simulink model "ASM_Traffic_A11"  (R2026a)
settings: Solver=ode1  StartTime=SIM.tstart.v  StopTime=SIM.tend.v  FixedStep=SIM.StepSize.v
PostLoadFcn:
  | if any(exist('dsrtsu_mdlpostloadfcn', 'file') ~= 0), dsrtsu_mdlpostloadfcn('Execute', bdroot); end
  | try, asm_mdl_postloadfcn(bdroot, 'UpdateModel', 3600); catch, disp(lasterr); end,
InitFcn:
  | , if any(exist('rtifpga_mdlclblib', 'file') ~= 0), rtifpga_mdlclblib('Init', bdroot); end,
  | , if any(exist('dsmpb_private', 'file') ~= 0), dsmpb_private('dsmpb_mdlclblib', 'Init', bdroot); end,
undefined symbols (not defined in the file): _to_, a0b2, ASM_BrakeHydraulics_DemoSystems, ASM_VehicleDynamics_DemoSystems, b98103fe8ad365046cd0, BrakeCircuit, controllerConfig, CPT, Crankshaft, DiscIntNeverNeededParam, dsmsi, FinalDriveAssembly, instance, MDL, ModeSignals, mu, Pos_BrakePedal_Maneuver, rad, RefSignals, s_to_rpm, SIM, SoftECU, Suspension, Tire, Transmission
libraries: ASM_Traffic_lib x135, simulink x98, ASM_Utils_lib x77, ASM_VehicleDynamics_lib x70, ASM_Environment_lib x22, dsmpblib x20, dsmsilib x15, MDLD_Utils_lib x10, ASM_BrakeHydraulics_lib x3, sl_discontinuities x2
(part 1 of 63)
PreSaveFcn:
  | , if any(exist('dsmpb_private', 'file') ~= 0), dsmpb_private('dsmpb_mdlclblib', 'PreSave', bdroot); end,
CloseFcn:
  | , if any(exist('dsmpb_private', 'file') ~= 0), dsmpb_private('dsmpb_mdlclblib', 'Close', bdroot); end,
settings Model: DataDictionary=vehicle_control.sldd  RTICANMMDATA=struct('GeneralSetupData',struct('modelroot','C:\_GIT\ASM\Demo\Traffic\Sources\Simulation\Models','generalsettings',struct('filesettings',struct('destfolder',struct('Name','RTICANMM_FILES','Check',1),'buildfolder',struct('Name','.','Check',1),'AbsDestfolder',struct('Name','C:\_GIT\ASM\Demo\Traffic\Sources\Simulation\Models\RTICANMM_FILES'),'AbsBuildfolder',struct('Name','C:\_GIT\ASM\Demo\Traffic\Sources\Simulation\Models'))),'options',struct('addpaths',1,'rmpaths',1,'addtrcexclusion',true,'cannavigator',struct('checkmonitoring',0),'show_usrtrc',0,'use_usrtrc',0),'advanced',struct('options',ones(1,100)),'MPSetup',{{}},'RTI',struct('Type','DSRT','Ver','4.5','Date','02-May-2021'),'modelname','ASM_Traffic','block','ASM_Traffic'))  RTILINMMDATA=struct('GeneralSetupData',[])  DSRTSU_INTERNAL_MDBS_VER=10  DSRTSU_INTERNAL_FLEXRAYCONFIG=1  DSRTSU_INTERNAL_RTIFPGA=231  DSPACE_VER=struct('Name',{['Aerospace Blockset'],['Aerospace Toolbox'],['Communications System Toolbox'],['Control System Toolbox'],['DSP System Toolbox'],['Fixed-Point Designer'],['Fuzzy Logic Toolbox'],'MATLAB',['MATLAB Coder'],['MATLAB Report Generator'],['Neural Network Toolbox'],['Optimization Toolbox'],['Robust Control Toolbox'],['Signal Processing Toolbox'],'SimMechanics','SimPowerSystems','Simscape','Simulink',['Simulink Coder'],['Simulink Control Design'],['Simulink Report Generator'],['Spreadsheet Link EX'],'Stateflow',['System Identification Toolbox'],['dSPACE APU_Table_Modification_Library'],['dSPACE AnalogSingleChannelLibrary'],['dSPACE Automotive Simulation Models'],['dSPACE BCE-HILBlockset'],['dSPACE BitLibrary'],['dSPACE BuildHelperLibrary'],['dSPACE BusLoadMeasurementBlockset'],['dSPACE ByteStreamLibrary'],['dSPACE CANObserver'],['dSPACE CANUtilLibrary'],['dSPACE DS5337RSimBlockset'],['dSPACE DS5381InterfaceBlockset'],['dSPACE DSMSU'],['dSPACE DiagnosticTester'],['dSPACE DynamicTrc'],['dSPACE ENGLibrary'],['dSPACE ESPLibrary'],['dSPACE FIUDS291ControlBlockset'],['dSPACE FlexRay Configuration Blockset'],['dSPACE FlexRayModelBuilder'],['dSPACE IOBlocksLibrary'],['dSPACE InfoBlock'],['dSPACE LabelInterface'],['dSPACE LibsDependencyHelper'],['dSPACE MATLAB Connection'],['dSPACE MATLAB Integration Main'],['dSPACE MatlabApplToolsSingleSetupBaseScripts'],['dSPACE Model Port Block Library'],['dSPACE Model Separation Block Library'],['dSPACE MotionDesk Blockset'],['dSPACE MultiSignalTa'],['dSPACE PWMLibrary'],['dSPACE RTCANModules'],['dSPACE RTI Bypass Blockset'],['dSPACE RTI CAN Blockset'],['dSPACE RTI CAN MultiMessage Blockset'],['dSPACE RTI EMC Blockset'],['dSPACE RTI ETHERNET Blockset'],['dSPACE RTI ETHERNETUDP Blockset'],['dSPACE RTI FPGA Programming Blockset'],['dSPACE RTI FlexRay Configuration Blockset'],['dSPACE RTI Gigalink Blockset'],['dSPACE RTI LIN MultiMessage Blockset'],['dSPACE RTI MultiMessage Shared Utilities'],['dSPACE RTI RPCU Blockset'],['dSPACE RTI USBFLIGHTREC Blockset'],['dSPACE RTI WATCHDOG Blockset'],['dSPACE RTI XCP on Ethernet Blockset'],['dSPACE RTI for Multiprocessor Systems RTI-MP'],['dSPACE Real-Time Interface (RTI1006)'],['dSPACE Real-Time Interface Shared Utilities'],['dSPACE Run-Time Target'],['dSPACE Run-Time Target Shared Utilities'],['dSPACE SCLibrary'],['dSPACE SENTLibrary'],['dSPACE ScalingLibrary'],['dSPACE SignalLibrary'],['dSPACE SpeedSensorLibrary'],['dSPACE StructureBrowser'],['dSPACE TALib'],['dSPACE UtilitiesGUI'],['dSPACE VariationHandling'],['dSPACE XILMapper']},'Version',{'3.16','2.16','6.1','9.10','9.1','5.1','2.2.22','8.6','3.0','4.2','8.4','7.3','6.0','7.1','4.7','6.4','3.14','8.6','8.9','4.2.1','4.2','3.2.4','8.6','9.3','1.5','1.29','8.4','15.1.0.5','2.7.6','1.3.10','1.12','1.7.1','1.5.7','2.7.4','1.4.7.1','3.7.2','2.13','1.16','5.1.7','2.8.9','2.7.4','2.6.20','2.9','1.78','2.6.6','1.1.8','8.2.0.10','1.0','2.4','2.2','1.5','3.4','3.4','2.5.1','2.3.1','2.6.6','4.3.33','3.8','3.4.4','4.5','1.4','1.2.2','1.4.2','3.3','3.9','2.3.2','2.8','1.9.4','2.2.2','1.2.1','2.1','1.2.9','7.8','7.8','7.8','3.4','3.3','2.25','1.83','2.0','2.8.6','2.9.10','3.1','2.64','2.44','8.3.5','1.4'},'Release',{'(R2015b)','(R2015b)','(R2015b)','(R2015b)','(R2015b)','(R2015b)','(R2015b)','(R2015b)','(R2015b)','(R2015b)','(R2015b)','(R2015b)','(R2015b)','(R2015b)','(R2015b)','(R2015b)','(R2015b)','(R2015b)','(R2015b)','(R2015b)','(R2015b)','(R2015b)','(R2015b)','(R2015b)','','','','','','','','','','','','','','','','','','','','','','','','','','','','','','','','','','','','','','','','','','','','','','','','','','','','','','','','','','','','','','',''},'Date',{'13-Aug-2015','13-Aug-2015','13-Aug-2015','13-Aug-2015','13-Aug-2015','13-Aug-2015','13-Aug-2015','13-Aug-2015','13-Aug-2015','13-Aug-2015','13-Aug-2015','13-Aug-2015','13-Aug-2015','13-Aug-2015','13-Aug-2015','13-Aug-2015','13-Aug-2015','13-Aug-2015','13-Aug-2015','13-Aug-2015','13-Aug-2015','13-Aug-2015','13-Aug-2015','13-Aug-2015','14-Jul-2017','14-Jul-2017','02-May-2017','26-Jul-2017','26-Jul-2017','14-Jul-2017','14-Jul-2017','26-Jul-2017','14-Jul-2017','14-Jul-2017','26-Jul-2017','21-Jul-2017','14-Jul-2017','14-Jul-2017','14-Jul-2017','14-Jul-2017','14-Jul-2017','14-Jul-2017','02-May-2017','14-Jul-2017','14-Jul-2017','14-Jul-2017','14-Jul-2017','14-Jul-2017','01-Jun-2012','02-Nov-2017','11-Sep-2017','02-May-2017','02-May-2017','02-May-2017','26-Jul-2017','26-Jul-2017','21-Aug-2017','02-May-2017','02-May-2017','02-May-2017','02-May-2017','02-May-2017','02-May-2017','02-May-2017','02-May-2016','02-May-2017','02-May-2017','02-May-2017','02-May-2017','02-May-2017','02-May-2017','02-May-2017','02-May-2017','02-May-2017','02-May-2017','02-May-2017','02-May-2016','14-Jul-2017','14-Jul-2017','23-Aug-2017','14-Jul-2017','14-Jul-2017','14-Jul-2017','24-Jul-2017','14-Jul-2017','30-Aug-2017','14-Jul-2017'})  DSMPB_DATASERVER_ModelPortLibVersion1=8  DSMPB_DATASERVER_DataServerVersion1=6  DSMPB_DATASERVER_DataServerStreamVersion1=3  DSRTSU_INTERNAL_RTISTBM_VER=26.1  DSMPB_ID_DATA={'800713',struct('BlockId','12fb6bc3-5111-44d0-a4e3-361b98a9a776','SignalIds',{{'026ddceb-0771-416e-9843-dcd8d1431538','61e2bdca-47a9-456d-99cd-a85121b8e8fe','d0b83999-293c-421a-8719-21ab1d67d0de','ee79a2a1-d570-4cea-bcdb-c9b139602f90','57ea1fa1-ca61-4546-b593-c63adff471df','4745b4fa-0f34-4fbf-be5c-f27e4134315a','de5a6e89-ccb7-4a59-b515-490b9b995fd4','ad253b40-3f00-490f-9ecf-d815cc0cc36e','cc49b837-b150-45e5-8f90-c3d0e2d27081','b15d69de-ed07-4862-a514-9609c89542f8','13fce408-6e36-44ee-bb67-08a7b0eb2fa4','0f4551f6-6300-456d-9d9a-57c69ec52a7f','d36d9585-c1d8-4a20-931e-65168d3abe38','f057ce8d-e313-4b61-85c9-b9b6cfbd35a4','6c11160e-2f21-4e5c-9a52-ebbb9f762535','e6450135-026d-470e-aadb-d378b73b5a20','d236869c-3852-4609-804f-fcde24edb3a3','dc22ee5e-8ec6-4b0e-aea7-12268f14ea36','758aa22a-c1dd-488c-99a3-602f258deef7','bc79a9cd-46f9-40fa-919c-8e2738391b36','ebfaacba-c463-48d7-b1a3-39c653a8c3db','464c7844-6639-4bb4-8711-079b53f28673','4c39bdf6-9afd-4077-adbf-78dbe8d90694','d3194eeb-2c4d-4fae-92b4-da69ec7b3ff0','1db3a7e8-3ac4-49c7-9bab-9691ec783862','90ff480f-e2cd-45c5-a9e2-c8c85a7416d4','f175cdee-a16d-4d06-b6b9-468792d9fc63','5037e91f-c007-4d18-9ed3-e85dcdcb817d','365a1b2d-a520-4285-8b7d-0710eb545db2','ad84fb44-ff2d-41bf-b3fb-6e536509c574','949ac335-20f1-4cbb-bd1f-899e13a3e7a3','821ab1d9-2030-4fa0-bc2e-dfd2cf9be3b6','b9c006ab-bd85-4d65-a229-7e38f2547f6c','555683a2-7050-45d2-912c-54f0995d7ba8','92371cf3-d090-4109-a430-860de30ac424','353c2b7d-88ed-484a-861a-3a12ddecabcf','5b259f8e-4f91-45a6-a068-ded45fefdcc6','01be563f-388e-4058-a34f-f6cfb35f92e8','924754af-4079-4771-ade8-70a8e93fbf63','6cf2dfc4-e3af-4f2a-86ef-faba7990cd7d','6c53c97e-f8d9-411f-9845-8d7d23140d3b'}}),'800714',struct('BlockId','c8c3f793-af41-48c0-af0b-d118a4506f01','SignalIds',{{'9a85b6de-5177-4fe9-a45c-5ce81acce6a0','07d402bb-9325-4ff2-835b-9988c7203a47','e23e99f8-e557-4f94-a0a8-73349e51b7d3','1e2029dd-c64a-4f77-920a-b53592f4df24','79f5377a-112c-44fb-95ad-b93421afa7d0','fab0e021-301d-4150-96e9-7c18ce36f7d6'}}),'800715',struct('BlockId','64fe778b-45c6-4580-ad77-0b0bfacf3090','SignalIds',{{'c4b7fff6-f5fb-46b8-aa58-6d02b0742f95','1b507cb2-f8a9-4150-a5ca-84f7e7defee9','0800db64-ae10-48a7-b8a4-d98403852f64','7b5be15e-1bb0-4f29-a798-1f0dfb3c643b','55455eeb-e67c-459e-83e8-a412efa38a5a'}}),'800716',struct('BlockId','110f2d64-38d9-4620-a52f-7bcb09150783','SignalIds',{{'378c6c24-c180-4551-b7dd-c3d67f95d979','8fbebc1f-626e-4f60-8692-ff751c91aa77','6c7a7005-bb3b-414b-8b4c-d96ebde91b51','fd069fef-3f82-419a-9093-61a227734c9d','43ee6e1a-a539-4eeb-8eea-2974459fcd70','b309ea5b-cecf-423c-8781-a1d200972b1c','ae18cdd8-d414-48f9-9705-1c32113b2bf5','a47b08e9-bc20-43f2-89f9-f6ef5b9b9052','d52309de-83ba-4b81-be00-3c772a7db2e7'}}),'800717',struct('BlockId','2899132d-e1ca-416b-8f40-193c3fe897ac','SignalIds',{{'0be58094-6177-48f8-a93d-65142150c1e5','0ecd58d0-6214-4a37-a63e-4304fffa59de','4e270858-0fe5-4a89-ae3c-f92717842777','7564fa9e-cfd4-4df7-85ff-40634c98855f','f1470ea9-9cad-48c1-ae87-969ea9d571ca','5b5bebc5-776f-4a59-bf41-42658f78f728','a2387763-f235-471c-8654-38e764b051d8','461d803a-6400-4d45-8627-c36525a15027','2aea000e-ed67-4eb5-bd93-f8c260051b4c','cbf9e4cd-e9c3-4c64-ae9b-53aeb7b537f4','2b8362d7-cb62-4e81-889e-7432047b1611','d9a94446-b01b-42e7-9a12-b8e6590ad696','8d0f7580-69d3-4b5c-9a99-fd9213d24abb','8100021c-0ed4-4fa9-8bda-2d5f13b5b25c','739ab445-ce00-41fa-b359-832193f86cf1','d8540c08-79a2-4101-8769-084a7d989adb','0456d1da-e15d-4f84-b42f-5f0d6692b1d6','05a518bf-3959-41e8-bc6c-520d23ad1964','a3f23e7d-f547-4381-9f96-2cf61720eb8e','b0dffef0-6031-4ae9-aedd-823f4c618df3','ad3989a0-e252-44d2-9a0c-04f71baba5bc','ceeb7a50-52ea-4ea4-9007-a364fa77e3c6','c1f783be-9b03-4e5f-bdd5-bb8170b1d4e8','c1ec2c99-3048-450a-b67a-74422a158205','92235c85-c9cc-4b2e-9e84-fcab8cbdacf5','65d7570b-7e96-4496-a46b-2ced650781d8','6a8ce03d-0951-45fc-b3eb-05c2cd91d985','a6c24270-e0ee-4c37-a87c-804f6f78e6a6','dcbe338a-832a-4956-b7eb-6f217ad8bffd','f3d6ffb2-cf2a-4737-8562-4466766efd81','e3fc5c7f-9c10-4ed4-b3a5-3afb283b4064','6d1ed271-15a9-4450-a3ba-f7bb57f64ead','a8ba92dc-13bf-4092-8674-9e191bb7156d','c7354c00-bb0a-4e0e-9409-06a293ddd3c8','0eb2deca-de7b-4d2b-aef4-e4c396decc62','1a679372-da5c-4f17-b380-c6a2bf11d2c1','9ab79166-e826-4110-a0c4-535e2d710ca8','390f325e-bb6c-4962-9120-8a4300e0738e','be43b800-7928-44f2-a4c0-456242549674','94810d38-2474-4cca-8aed-c3c732d73dfb','a3c555d4-b57b-442c-bc5f-42b549e0ebdd','fa686c6f-57fa-4a19-8654-6bb0d89b9d8b','317fafc6-aa92-42fc-af4b-7e632b8dd6cb','42f758a5-2c9e-4e81-9e7f-7d05391bf3b4','95628c4c-8a2d-45d6-9031-c67e967b97bd','053040ee-7507-481d-9488-55c16059fd65','321ce886-d869-4a8c-ad53-a1182d7ebf7f','2f696ce9-8e82-4494-85b6-6edf41a524ba','96c19483-5db4-47db-b22f-cb8f6c71aaa7','4ab31462-1fe1-425e-9686-6c57800097be','abf784ea-ad12-4b9b-bc2e-530352b16490','38c309fa-99f7-46f8-8d6e-2b0e652896be','e8acec3c-5d72-4d22-a694-701a6e4415b0','1ff94e3c-5fa0-4134-8bb8-33777bace64e','9fc01bdf-7a2b-401a-9f97-847a1bae8365','382a0f0c-2480-4a75-9d5e-ae6ebdcc659a','4eb20648-628b-4e6f-ac33-2eeb9d126ccb'}}),'800718',struct('BlockId','c7b5bfe3-a6be-46ec-a50d-4aab3ffc24a9','SignalIds',{{'deb772d2-6c98-466a-af94-833c1e8c6a36','cec82f56-8cc7-4b94-b67a-0596894dbebe','6382e864-8515-4680-a048-db954d71ab26','91e981ed-2272-4996-ad40-8a28f4d6dd53','9d667ac4-4e72-44d2-8b3f-72ed78a704bd','b18fe58e-af28-4bce-959c-12f7f85ad0f3','3aa2c131-9c84-410c-98de-2fe01e4a908b','35507932-4bd5-48e2-9485-b375285d832d','cd5b9c3e-56c1-4d2b-9a1f-945395cc32d3','24eebe62-153d-4bce-a518-49c16cde84f5','4305de8d-f825-44f6-9ca5-0c7611fd522b','17e29716-ca54-48d0-bc62-5fe9f3434ca1','cd3b7b0f-c36d-4cbb-9379-f81b2c6784f8','58d80150-ba28-4376-9565-4f54e4772edb','c576d0a5-0790-4567-987c-cbe91a75f0ba','50664475-5b64-4e66-9f4b-73bc2fea1a6e','aac5ca77-fdc8-4e25-87c7-90ed104b35ab'}}),'800719',struct('BlockId','fd333250-5108-4bdd-b217-05742883b635','SignalIds',{{'fd6e4402-dbaf-4d1c-bd82-13425e573e08','80cd8a48-d5fe-43c4-94e8-1cb6116a8ed7','c93f02f4-8690-4b3f-aacf-dccb2e469f89','97a0d73a-2704-491b-baea-065e5044d9d2','84a2e8dc-aed6-489a-94c8-65c6b07fd9b8','dfadd777-133c-42ac-820c-b33d6acf198f','c486474c-f3c8-4087-9f03-9d730f82c385','beba5407-f372-4db7-a348-241e24965918','ad25fe6a-7c71-482a-8ce4-10e2b2982753','277316e0-b6ae-46e2-b77d-e820d153e69e','1f1ccb49-e040-4775-b555-ae961c45c1ad','f1e14c28-6f99-46e6-b62b-c3d342fb5443','91bc19e6-da3c-4265-aeed-a1989e826b66','47a757e7-3497-432a-a330-11ddc874cd64','8d6042c8-cd6d-42f3-b882-ae0739e92277','4cce8199-ae31-46ba-accf-bf53829b41f1','5635eaf9-a30a-4fc4-ae77-4cb5eca17a9d','ee61cb28-d577-487b-8d44-ca6116171fcf','e7ac0723-c0ce-428c-8c8c-067eeb8da74c','d1b53615-1e53-4ce2-b64f-38a5f7733f09','cdbdca06-6486-42aa-b430-cb4a52eea665','850a5dee-225f-478a-9581-615a2f48f7ad','854c96a0-0707-4b6b-b6f8-0a183b00e44e','b51f722a-63c8-4799-80f6-5869d1768c86','afacac09-78ed-4c28-afc3-caf5182c97e4','3838c120-da0f-43e6-8c82-f4acfe70f498','0ec37172-fd37-40de-a1a5-d592bab9638c','f6432d1b-9c84-4f2d-9c11-26b8895372d0','88cd5d72-dcf7-4fa2-aa1c-4defdddab07e','9e3d05f8-118b-44d4-bf73-9541a35eccb6','47c50691-23f2-4614-8d16-3486ef70962b','df1199db-e244-4ea3-ba3a-6d95e1d3ab35','d0e15ae8-1f1b-4aca-b5c1-25fd3bc4d7b1','943c66f4-642f-4813-83a4-aeced7a93800','a414337f-60a5-451c-85a6-1cf67a2bdc2a','47656cf3-7131-4a8b-8897-3d4f5ee504dc','19df50e1-62cc-41c2-a1ae-8a30072c1769','6313e6c4-800c-4bc6-b483-562a296c6696','253d101f-cf3f-48bb-8256-ca9e2c176994','842ccb91-7488-4424-a1bd-ee0dc5452e02','edfb4f2c-8887-4268-896b-d3d4cf08511f','be61a72f-860b-41f0-ae5f-29ebc26172cf','be000a67-2b4e-4015-b53e-1fbbf3a008ff','462755d8-e6d8-4a64-9626-426b47122f26','82c58b5b-69d7-4d8e-b402-7f1b4c1a700a','1e6d3f4b-3b03-470e-923b-22159f6cada5','5f049c30-bd46-49c7-ac48-7e1f6fefb530','a0e0b802-6f7f-49b7-a429-c48ca4d4139e','1281ac42-8e28-42c0-a936-4005a211601b','9beb0e9a-27d3-476a-9d13-99abe4cea843','f53d3867-dbef-4261-b1c3-2b4dee163be1','ee2aa355-4a17-444b-902a-772860eaddf1','32460b21-dccc-4b01-877e-a94aaf934646','863063ab-8cc2-4a40-b442-f9966cff8d6e','83f86310-1a7f-49e6-afc4-440052af8f12','47d5607d-3f4f-46ab-85b1-751519f5b805','08ed226f-598d-4aac-861b-044b7f32584c','4bd63bc5-4130-469e-8f22-d01f9f4fce98','ed130744-95a8-4396-98fd-6fdf7b74c868','d25515f7-636d-412b-a108-6469ece34014','e0a9f995-7fa2-47f3-a847-f9f484ba4f2c','b862dec0-72c0-4713-a690-404fc8b02f29','c3bb2c82-685d-49ae-b6af-b90687468879','afbaa59e-7f77-4310-971c-bae7947abc48','90602b8e-bb8c-4b0d-9b2b-c62ce4fdf7e7','1c856c8b-b541-4516-b46b-1f3d62cbbfe1','7cc261c0-4f47-4e61-8dd4-d78e25dbdecf','c7bc511e-0b65-4e98-9c9a-920064cb6b63','bfd1d56d-f13f-4e5e-823f-952e754dbd0c','82de7653-b024-4c13-8012-f38d758e9954','2b4044e1-44f2-4903-950b-be8ac8baacaf','0dd165a1-5364-4028-bd1a-b406b00946c2','2f264a39-d831-47f4-96bb-f9fe5ff30a53','9df5b4b7-db8f-4bdd-b4d5-9d6a9a0ffdb2','1a66a4ee-350e-4c2c-bf40-f022062406c2','77a18b2e-c672-4761-91dd-6eafa4e19102','12d51f03-4dbd-4ec6-83b2-f715a521a52a','7bf7b22e-517c-4b95-b2bf-97bfc99264dd','add68492-0910-453d-ab19-c30bda99b2c6','cbd58389-3dea-48d1-b9e1-406211fb2dab','e50a4cd7-600e-4355-bb15-3c094bcc5ac1','3a0447da-a263-4f93-93eb-0e9b9100edb0','912e2f1f-6f47-44d8-adcb-1b8177648d58','e486dd64-d6e8-437c-a6a0-b199f2efdb0e','d2ee6f75-3cb1-4eef-983b-ed71a6d1bb38','c1952aa1-b2a5-48c0-a2d0-942ec9e7f2f4','49bde967-5132-4542-89bd-c4654eefdd77','3be74dcc-f43c-45cf-b54a-b5c65f19a43b','818406ab-e94a-445d-b1b5-ba61124e00c4','8f71f621-8c70-4d64-a2c2-b488647126d4','4da05b13-dc65-4e7c-b1b9-878991124cbd','6e83efe6-c8f9-4231-92d4-b4d7f0668546','69993996-e1d1-496c-aca1-69ffe8fae1a5','84fc7653-5de2-48aa-8e1a-968f1166a742','258a0b8e-5f88-4752-9ab5-3c0b8ebda0b5','441ae18f-f8be-4dcd-b94f-7ba9930a13ac','21dfff82-3c2b-4ea9-91c7-dcce8ece5997','346f0f1d-f939-4453-a2d2-0dcb996e0a1e','a36adb97-89fe-4899-a265-6520c71b3ff5','813f486c-74f5-4eca-967f-6c42063ea4dd','c4d42689-f4f0-4b6f-a38e-f84d5d9356d5','b6f52c18-269e-4fbf-8d79-b3a8502dcf1d','be3be440-49a6-4e5e-a8ea-e101f1f97e46','1443e3c7-0b66-4559-9d5c-022bd6fb1413','3619d79d-62a1-40ad-8798-8aef318fc3c0','ccd1bc00-75bd-4940-86fd-cde09b68246b','4897e56f-50bc-4408-afa8-8836e69b4214','2a747099-ef0f-49a8-a673-c9e2bf0431a8','2a05c281-76dd-4b18-bdcc-8b0b1623de33','8e8b9e3d-9da6-4c91-ad97-da351e7c5ce4','3aa74a25-b846-475e-b85d-2bda7118e9fb','36e5d7cf-1e55-485d-9ea5-607404581b83','6e9c588c-5111-456f-8df5-7d28f79b85fd','11f87df0-b446-4532-a0da-a61e3f519a1b','eeb7ca53-14f3-48d3-8cbd-30d53393f24d','15cb62d6-efef-442c-9095-4a4daf8331f2','571764dd-0a10-437d-a524-f0b9ab7344e5','8b504bc9-b5c9-4e82-b1fa-78aea347ec15','998dad1e-5600-4381-ab22-e7f3f524ae7a','662aecf5-3045-45ca-b11e-e7d87e8d0b8a','b10085a7-b175-4d8c-b90f-2bc7d40414d6','f4edeeab-2a70-406a-b919-7fdbdd2abf9d','37caa2d2-32f1-4563-85cc-686b833a5474','f4833482-eca0-4dbe-8fa7-2a1e94c23c99','e51f2174-4775-4a15-a086-b4a7f7e75b6b','8d7a3b7c-fd97-47f2-8c27-22f6e203736d','e5956908-2186-4f10-ae9a-fd057fe70ff8','721d1792-f1e9-42b0-a3a2-0e3fa8e0e821','d2a202d4-6127-4e89-935c-9d92cdd87736','386fdbd0-531c-494b-8426-924329178d82','efe7a87d-9b97-4251-a568-6f0ca7f4e92c','1f7fa3b9-bbd9-405e-b404-8a9e18586bee','432e3bed-77cf-45a5-85cc-11e334fd07f8','86045c54-912a-407b-b67e-f78922ce536e','457cdd77-786f-48ea-b3b2-c3e03235aa0a','633e14cc-c11e-4ac1-a483-775611aea1c1','a258e7ad-81ee-4dea-b8be-6e7ac4e44621','4ef6a072-1e8b-47a5-b341-a5dcbcd8cb90','33a3ceb0-8ab8-44a3-a3d2-f71013987fea','c36f3052-c68e-4376-b40d-ddf2055ae487','75d2ad53-8848-47bc-b5d6-a7e0017612c5','bd5d9453-6739-4499-981d-84dd39093b80','969f387d-3fc8-407c-a5e5-028362e5a95b','f11fe3f3-e9fc-42ac-844b-205184b71153','499e8514-fefe-4d7a-b40c-ef24d59ba918','a8201869-cac4-4380-a59b-e6c9f75760dd','98eed4a8-86bc-4747-917b-86404f1357ed','e289c530-b7de-4f7a-959d-0126ecacaf5b','5e5aadde-87cb-43d4-9746-29a9e6093a01','eb12c2ea-8f65-44ff-b461-5fd33f643dd4','bb210c61-1ec1-4936-995b-6bbfc57ddf98','e18cb670-c569-458d-978c-40f8ce8be5d4','4fbc0806-ca61-49f6-aace-fe0dcaff62a6','e7b2d3a3-c8df-462f-baaa-a2d16ec68154','f460289b-3dc1-424c-921b-29a4e305af97','f7d7a98e-f960-4832-bed6-be5d87bc3939','ada121aa-b9e0-4352-af98-831065332c99','384a259e-8ab7-4f48-bcc5-2d9370d1f415','41a3b8e0-6640-407d-bac0-c67ec7bacf7f','76e3ba12-398d-4d52-8e72-77b36df0b8f9','cbf1e48a-45ea-4ed2-aac2-f30a6de77e52','5b48e4e9-cb2b-4d01-ad8c-9e091345c2c7','8f53c525-7b72-43d2-9700-c7f983d8bedf','1cc60d1e-b8ae-4cf8-8851-0c49bafae1ef','be881860-d9f9-47b3-9d26-2e8339e236fb','2f5214f4-3645-4631-9005-571891b6352d','2acd13c6-dc04-46ae-bbb2-6839e982ab9b','9c40bc30-58b7-4191-8583-d0a20298e448','673b273c-3b84-4498-8285-a0a40c19a0f4','f19513a3-3d55-4382-a04a-5103d5267d86','5b5d4cf0-5436-41ce-8909-db5899b0366b','34adf297-cc5d-493b-9e6a-f695daa8b49c','3ed04828-0fc0-4e22-bef2-0a837b1a85e6','10cc9fe1-d523-4eeb-b681-c0c9e714530f','651a801c-6def-4724-9352-2a0d2f461e9e','0df446cd-9d88-4826-bffc-e9c9dacefbfd','529d7a46-f3fe-4bbd-ba1f-0fa165edf0f1','839c4579-a867-4396-b3ce-b6ac5267bb63','4a4e2f74-833f-4f7f-a54b-0a013ee938dc','85878658-3eb9-44a1-ad3d-539db9b60dfd','b3bab6cb-b43a-4861-9cb4-d8e7e4b2477a','9e08f04f-1cd4-4178-acdf-28e3ba30a904','e170d6ef-c360-41ca-b395-23487890b9ba','26eff205-14b9-4985-b337-2ee8592d01ee','c5bd0156-31e4-4237-bae7-be3fbabb6203','19a317f3-6d6d-4b8d-be7d-2f7dd3f41750','124aebf3-3ce1-4170-a17f-7ca68554ecab','260553de-b45c-4d7a-9ccc-678cba5c894d','c193bf19-d2e3-496a-b007-3e21fac56152','cbc4fb28-7ad3-42de-b3ee-6295ec2f5ed3','28f39ef9-8949-4eb7-a170-43df15bf335d','61054bc3-cff2-4e79-bfde-bac599f810fa','e865ec6c-644e-4526-b712-0e2c4af0429c','32d97da3-463a-4a75-9f72-02b74bdc2bdc','88c36d39-a5f0-4d09-9904-1c7d2863a1e5','b034d8fc-249f-4dc5-92b7-0e3f3fdddb16','55809439-d5b0-440e-adf4-415722c7ff7d','ec6ba6c6-5833-4612-995a-d48b47c2f1f1','b6a9966d-13f7-4837-aa64-8ac9eb77e9fe','1d664ff5-9564-42f5-86ce-0d8c55423f0f','9f619f56-85ed-44e0-be73-a9b7045679b2','68285cc2-83af-4a99-aa80-754e09911ae7','11d1c7e3-e8cc-45ef-98ac-71242c47fd69','e3c649b7-6571-49f0-b0fb-7ed4a441295f','11e241bf-760a-480a-b056-0d8ea1b83eb2','5438b643-3610-43a0-b3da-962e8ccc3a6c','70645b38-5664-4bc9-820c-6fb34a07cf55','bf395dbf-7dc4-4a31-bab6-f5f2d09649ef','9b6ebebd-ce58-4762-809d-f61da916c82c','8e5c654b-aa01-460e-ab69-b31230631c49','5b25f867-2790-40d7-833f-efd4b524b300','d29247f7-3ac8-4f63-91df-421bb2412626','ea999d2b-b741-4245-97be-0568eb343541','ae6ce583-3c9d-424b-bd65-be44f01e3fe2','dfd20957-1c86-415b-98fc-03254081b7f9','d5258cd8-92b4-4d96-b282-a49a7bb033a4','91e5d8c9-c3be-40af-82a3-39f6fee7fd72','ade0190c-86e5-48c4-8cbc-94be3d179650','926c42aa-9323-4532-98b6-cbace0f916cd','815ed81a-3c7d-4cd2-8ddb-729019ad6a5d','96882bdd-5ef0-46ff-9e86-5f86cd211018','1b29f201-1d91-4a69-a201-e625071d402a','132ec7eb-3cb2-4b84-8dc9-c1b60432f37f','fefbfcdd-fb77-4e3e-bed1-dea215a465b2','ac8187d5-70a3-4e9f-9fb0-449d0fd95455','a2468ef4-b5e9-4bba-8079-90fa4fe6ba9a','3a481284-d6e4-478b-815e-e8b7ee39b804','3f743739-8eed-4907-8e00-1e69c5f7a069','612a172c-d71f-4bd2-921e-ef8122322753','b39b0281-6a32-41cb-b61f-fe1c48652b5d','3dffdcde-cbb2-4b30-8f10-a79bfe7ac8a6','174a1577-cde1-464a-bd92-78c85596ea9f','a481522d-6416-4477-8366-d162f36f854b','1934cf53-bc85-44d4-9834-32f3b40f6723','7dbf76fb-682f-4e30-8ffa-a8964982cd31','460b5546-faef-44c2-ad2f-c8ec09c213fe','3e8e108d-8057-471c-8f27-6384e05eb336','4d6530d5-13d3-43f6-ae1a-ae00959e2feb','5d78849c-472e-496e-8997-147484f6e235','d5e3f857-844b-421d-a89f-de300873403b','2467ee71-e27d-46be-92c8-98b34bfcf680','08b1e42c-5a93-4422-8a26-fb864646bd3b','a7d2ec64-2af0-41f2-b7b2-76e754680827','06e7b93c-173c-46c5-8782-7ee187ec7881','a95e196d-d174-4334-ab10-6a04bd9294f9','52cfe45a-e2f3-491b-8eaa-420863bfcb65','a68fd712-6029-4f60-a22a-817d7a30cefe','625a9e93-f1d6-49e8-aba4-534a3637cc20','21c01b24-e09f-49b9-8e5f-1df61369280b','19c3c8ed-e25e-4cdc-b3a3-a4c88ae3ec08','a65ae3e8-7273-447d-a9e6-6b5ab4056b67','3f691ee9-f7bc-4257-9b4e-a82410e6b361','54005e20-c57e-471f-884c-c5d1567287bb','d141b19b-de14-46ec-b875-aec65db0f863','721ff134-45db-4ce2-8195-3b47226d2168','1b7dddb9-c9a2-46fb-a905-0b22176f1b56','f8d458d7-a8fe-4c9f-b51c-513ce92f8f58','96d248eb-6503-424b-8262-2971b27663bc','5c543db2-8f3c-458f-a87f-88d3ad34e75c','84978c9a-d204-4ae1-b5cc-def3db43d3de','94c6de6b-506c-4e12-86a5-8c30c0bd3d29','52543c73-8ee9-413f-b8c2-c1cce940dfc6','4f5281bb-b87e-43f4-bbed-594e1b06c856','4b3a4b30-979b-435c-aaa6-d0336629f976','23505fde-e56b-40ce-8d76-a8d68cfe1ef4','639e0dd6-03b0-4dc7-8cd1-c7f7b0fe6c6e','42fd96c8-5980-41ea-a0da-b97ced6595f1','88f66b5c-1ac4-4559-b31c-77f19b1cd8a5','b69ff814-aa66-41b4-80d9-93d52559bfdd','d30870ca-c7dc-4765-bd62-b1760f9487d5','704b5f8e-a314-425a-82d4-1f88d8338332','2928ac11-c1ab-4fb5-8d7f-6cf1921549f2','b6ddf3fe-def7-4b87-af32-d46497b5f280','26f65cca-2b8e-40a6-8d1e-77532426b3c5','9f9a1bf6-5e26-4379-90b4-cad69f22f46c','52a7ff97-c3b9-4afd-87d0-5d507a16b43f','ea85144a-0f6a-4e60-b347-f0847d464682','e7406b7d-23d8-469c-a87a-20dc16cce629','09d122df-62d9-4fde-b517-307dd7f247a0','1af483a3-5dba-4e87-946d-edb9ff10d952','af5f28c9-9b6b-4c54-83f6-83efca44db43','358c0144-6bca-49f4-856a-505f0005ead0','dae519b2-8fda-442b-afbf-a57256228e4a','cabdeb0c-fd14-4480-809e-f8bd831530f2','3753778d-7701-4191-a108-f95c031e210e','050dfa84-9801-4a77-89c5-4e18861e0eff','0574453d-4f79-40d2-9295-436a38ea6fa6','33ae45f5-1b0e-40c7-9e1f-6a891aaa99eb','f5b00419-736b-4db8-b323-33488acf2321','e31680d3-85f7-4475-ad81-714e9c77096d','559a82df-326e-4ff4-a954-25b8ea3fce8f','75ecf84d-9e7f-4f79-b650-def95bb1dc28','ef02442b-a3d8-47e6-8210-b02af6b4c3a9','33c85bf4-4e4c-46f7-8153-16ca227d767a','8cb07083-0435-4e69-92f5-dbfe701ce639','69d9bb28-dfd4-4fad-beba-5bfc363a8f37','cec7bdd8-6b8c-475b-b5d9-60afa7ae3192','a2757570-f0e8-4064-9904-47ad6785786f','5098ea65-99d2-4ab5-8f42-68659c491850','815273cb-95f9-47eb-845f-8c26e9f27b18','11638e5c-c925-49cf-8400-a294f7fd0d4c','e38f8c63-aa2d-44b6-9217-b7627d8b694b','5a27cdf1-29c9-4958-972c-50c8479d48f3','9547b75f-550b-421d-9209-b17db36a7b38','3936fd79-6d0d-4670-90b6-6d6771523efb','39ed78c1-b78d-44df-9467-147dd44a331e','28336012-56ba-4a27-9f6b-8072957e2ab4','c7f345cb-a5a4-456d-aad4-d6ce6d38a8f9','63c5fc1f-843f-4e8d-80c8-668e3fb21a1f','8f7539f1-06af-4626-be0a-9bff69a1368b','a1ac348b-70ee-488d-9aae-dedf7c64629c','49873e84-badb-49db-a2fc-12f790ed48af','e49b3b6b-9177-4785-bdaa-9a55e5bdce1f','6ba9c8c6-00d8-4aa8-a682-db91d3d5eaa7','dc60004b-64b4-43ce-b552-6a705e29ad2b','f0e9b7f2-9a67-4c00-af33-0281125f96bd','fc18e226-c085-435a-9c7a-d7f67332d7c7','9260f897-808b-4c02-8893-ce7a9502e88f','0ab0c39c-faf7-4ef1-8f12-0417589d5025','7b759374-9407-4340-a5e9-1fe8ba3752fd','4e13c8a7-6ed6-48c1-8003-99e5aa7c29b6','ac17a9ea-49da-4036-9736-9cbed29610e8','0d378965-930b-423f-a840-0c051819108c','ca6cc074-cf2a-49cb-bda0-1d1dcc853518','5cc8784d-dcfc-4b38-beb8-846b34311f7e','71c3913a-d9b4-44ce-8d18-57e2e0349ede','415d9c61-3908-4b19-afed-0ec2babb0b3d','933897ad-7807-4fa4-b984-50588024d1ee','9523dc80-8cc3-4e1c-94a8-7c554f4893ab','3cbc7db7-12e5-4909-af7c-ac14a16fe7c9','ce8eef0e-065f-4f3c-bf40-8320b55ed4af','086e1f14-f97c-400d-a71f-65f8443b83ee','464499c0-e684-4365-972c-478dcc5b0a6a','887bcdd5-372e-4a6e-ae1a-156a22e91639','94534093-ffa0-4f6e-9caa-344ccca31f9e','0da13333-6bbd-4009-8d66-75a409e4c373','0f040adc-e949-4a2c-aa12-a9963cd99090','5cc8d786-8e7e-4a80-935b-2c403749ebf0','62e31b95-3767-481c-9e26-877e8512715b','494500c1-2293-4f5d-ab5e-e0e711e0a481','ec62fb6b-6b7d-4362-ba4f-ca9d3203c8d5','dd504bd0-6ac0-48ac-9941-c1b8393a5d80','131b1c51-8d29-424f-a52b-b7486b8963eb','481e62ca-99f1-4a59-b2ed-f283d2c6115c','d1f822e7-e193-4105-9944-5ef88c09e16f','343cf794-e84d-4df2-a0e2-cc3cd0e5bec9','93f4156f-6ec5-4502-a0fe-ef5556cb76cc','b0c1ce3d-dfae-45e8-8454-8c489cc21e98','913c5031-27b6-4f17-ae89-80ffac7b34e2','948598ac-00e7-44e8-8f45-e84c6233f640','2768ec05-b70a-4594-9019-d8e51a4c3cd5','7e106a19-98c9-436b-af0a-07a9add7d568','a37c1230-fe21-4076-9870-b4e928ad5f9b','13e33e09-6991-4b75-a839-d00d08231ae4','b29ca0d9-309b-4e46-a215-2b21a81b760d','0e80f926-54fd-4849-aa5f-4e57b625b6ec','b895fcc3-51cc-4144-b4ba-c47590b36f3f','b6c7ae05-c5bc-488f-9714-c24fe9239592','dd7fab44-de6c-48ab-a299-b63839da8efe','2c851ad3-6fe2-4adf-a2c3-441819fefdaf','cbce9f07-5814-42a8-9bb0-e1bc65b8397a','4fbe92a1-e813-4a5f-826e-2a64377b21dc','08b16216-c2c6-46b1-8a8a-b5fd204d226a','d80542b3-d744-4aaa-bca1-bd5c218c6c28','ed3860f6-cf92-4352-9611-615aa549b8ba','ad39b900-aa89-46d4-ade0-88ca02801db5','835dade4-ed68-4822-9f0f-91d4a8bef7f9','a5f4612a-c2b5-4a1c-ad56-601dd7e5e292','434e5f50-b582-4e7d-b369-fb3770492bd6','cb6a7a85-a645-4205-9f2d-680836e5745f','dc9bacb9-a556-405b-81a3-cb1e86afb47d','26e9a9aa-b2a8-47f9-a33e-5677781dde07','6c80ef6f-aabf-4057-a976-4d61c6b3a064','00d13d95-38c7-47db-82f4-2674a90fa117','ce205cd2-3e23-45c7-8998-00463b8a5e4d','eacbe410-69ab-453a-aa15-cac43d24a0a2','f6da750a-f36f-4cb2-ad7d-abda2f03264b','2291bd63-7118-43d3-83b3-2de0538cfaee','b58d9e44-1610-4252-86e0-1bf77d645639','6154ec9a-a5ac-455f-80bf-851aa4c895e6','5db1febd-d804-4f89-b857-57714f040b5d','7e5ccd30-3da5-436b-90ad-6b18dcd7161a','0de7d095-52ba-4304-96c8-d2e1d9610f6a','dccf3787-2c59-4b19-8c6b-bbadfe2e9f60','68064b1e-7655-45ee-97a3-4e70dd6576dd','849eb62c-63d3-4039-adeb-70b9d37fb488','13b3e6ce-f212-42d3-bb14-f7c00525e8c2','cc45035a-c2e1-4e60-9cf7-fcc914c06f13','b723968e-9ced-47a4-94c8-4ff626121c9a','0026eb22-f012-43c8-9a76-e8f5ae24bdbf','e72b21b2-6adb-4e80-932b-a04864c86b0d','98037a7f-b972-4c57-8fc3-2ed3053acdf1','7467eba6-da3a-417b-8b03-86913cb536b1','c4061991-c600-4b56-9c1c-8ae8c0db4fae','795c7cbe-7824-473d-a588-36b3ae1f35ad','72a6ed99-4729-4450-a69c-d529d4bdec71','1fecf23f-5df2-46be-8767-ba6d6f373f5b','403079d1-394f-4ff3-a41d-e4773b4c7961','432b9954-0769-452c-a5d0-e2a4b00f818d','2b08d00a-ff03-46d8-92e0-60ddb81dd1ec','25cfa554-830d-4b41-b47a-f922ec4331d2','77e0fb02-ec46-4100-bb0e-5c21f8f17d49','e674ecea-bdf2-44c6-b4b2-274dbbc24771','0400cb1b-6dbe-44b4-9af5-d6c6de8fff09','d9d8bb5f-88d9-4283-9fbe-750fed3ee86b','42ff59f8-bf2c-4b68-a505-dcc533f0bf83','cff205ba-a570-4a23-a12f-b3b1416edbc9','815e9bc6-f30f-410c-bada-7e417c88ca9b','6778aeff-90d2-49a3-9990-b37597950d6a','585918bc-fca7-471d-aa16-21df91b1e575','5b1c5a9e-292f-49e7-a123-aad2504f6bec','bde42318-2833-442e-b230-b1aab8da44f5','9d313b57-3f05-4537-b910-8d7529b9df56','c0bf9cb6-c74e-47ef-8345-69b83a4390b7','2052d4bd-d5d9-4cb4-8fee-b926cca08886','59b73606-3ef5-49e9-841f-9142d51922ee','34e23f41-a493-4100-b89c-08151648add6','4e9c1654-a2b6-4ee0-b051-28ffe9d83236','5d88254c-d548-40da-9564-2c3188f97159','994ba359-9a61-471f-9029-49bfc628e2a5','aa894a1f-0197-4503-b331-0a5869de3b51','f826c54a-bb23-4099-8bc3-ab38dd2e865c','0b6a15cc-de93-41ee-8a25-d5adca07eda0','f111bab2-14a2-49d1-b9f3-cf10c236a74a','c6780fce-b536-42fc-89d2-6fcf0cb4d612','9e451274-9716-46df-9152-1064805ab97f','6fb91ff1-da78-4def-91dd-787ec10acabe','a457fb63-f8f5-4ea0-8308-e6f0a32af7c4','9b8db872-6f29-4474-ae6d-21a2f0d965de','b684aee5-ece6-4ce9-baef-4c184bec5b46','b7e2ee6e-5797-4de5-be77-8a7a2470d2ea','459e31f1-1048-4237-b65e-53a682c496cf','007514e5-20d3-4be8-83e4-0c12eb58cb58','678b0e61-55ed-44d6-bc51-a73fa6039c8b','fa391d41-17a0-4380-9158-d5bc18502f71','23a93a4d-f561-4313-9bed-60bdf5532ba2','adcfa876-cd79-4b10-8cea-4a7dee1e1b6f','b96271f4-0769-48df-97be-e6aa85f64d1d','00f087cb-f29e-4b5d-885f-3d0712d563b6','3f8d2702-acef-480c-a245-d8665783d58a','9ff38e67-63cc-4a63-ab15-e8813ae91844','58838c44-8815-4161-9fb8-09ad3d94ab57','65737870-1d0a-4325-9022-82e15d4df7ea','4c56db61-31c1-4153-a5b8-0073a4d26812','f1caf4bd-759d-4971-91df-283762315c2a','651850a8-2063-41f6-9b0d-b42f8c80eb17','44760097-d096-49bc-871f-cf942a62703e','53032c65-7241-4335-bb3b-133c6deba1c7','e901a969-3399-47af-bd3d-8d14acc49eaa','086468a9-dde6-4534-af02-75149b6a36b2','5451482c-4aa0-4c71-a23c-110b85a13bd2','7074a757-023b-4f0e-9560-5f2e122d4106','fbbad7fc-6304-429d-8fda-8745d6e71865','6b5b75fe-41e1-44c2-8758-d045c1ca6c3c','d7103f76-0f32-4732-8f5f-9d112aee083e','0bb65106-778b-4795-82e5-ea5332a27199','0566b4ac-d7c4-4ab9-89ae-cd72fc268dd1','3edcf7ea-d625-4730-ab9c-92365d346485','4a9bebdf-f287-4864-a024-c7aa97acbe93','8785b728-6ce0-4fb8-890b-0da1f1171118','8b0d478e-4531-4204-9114-8c8af00ce770','bcbcbe8d-4751-42e1-9f8d-5489ef6faf4e','b3d6c537-45eb-4f29-9815-c2c0fda43e1d','29a4883f-2662-4f0b-b175-94faa7894996','dbd6aa14-0b22-4f80-9140-1d7e159ca164','3b7918f1-0943-445c-8e4f-05dae4e7becf','6062afb9-8f78-4364-bf1d-f789c0c511e3','021f4b46-bb06-4963-be58-221869a56d5d','7de15bc4-e126-4750-9d36-fe9d7bd39a2b','b1959591-2556-4c2d-8ef6-ae6a161e5f66','3a2f5d83-d28b-49a7-bb9a-4266fd82e86d','b7eed133-2659-4774-acca-72a358f93f36','c9d9a9a2-1f9d-4edc-b930-a889e41f6ac6','08f5a3a4-94f5-410d-80d9-f01f13278ab7','abbb1ed0-df06-4eda-83f6-670e580a635e','85625479-f35b-4bce-9291-d5fea5685085','c22d387e-0389-4ea7-9619-2fafb12de9da','a3b726f8-5419-42c5-809f-ac58730b54ac','5c9e6f33-45b6-4b48-be53-07f07c75dc60','18186463-8bbe-4d22-b967-a357177b8992','c5d313d2-7fb4-41f6-ab7e-970f642bf661','43cf0c75-731d-4427-a607-ac297c9b04d4','bc688c1b-f79f-4537-bd6a-90f7f70258d4','2a824880-b617-4812-8fc0-e79c36078579','5b40b02f-f483-446f-ba8b-9c0590a9aa52','3ffbf29c-e93a-454d-afd1-15d0cc75740f','bdf917f8-f31f-4422-8612-47cb7fea4c94','c159c3b7-58ff-479e-843e-739019a2d083','77b79784-c881-496e-bcae-3456f8be2890','7d515c2a-2100-4a18-bc20-ca36e8d1fc05','db67a7dd-5c06-4444-b504-16e4c6056ba8','78ba1537-dc34-4891-8579-029b4bda016f','8cdb5d89-5bea-4dc3-a8b5-5fe7bc447037','fa021e40-1544-4157-ac51-21b23ad30aea','3eb8862d-80cf-47a9-8631-9cccbc06d8d2','9471ca46-c0e4-4fa2-882f-da219449c3ed','2c13c50c-ebd9-4f63-84ce-e5de77c0276b','c285ad12-b145-4e88-aa97-6fc877156147','6df5545d-1ead-44bc-be4d-6a4b444f096e','9e72cda0-2686-4aa3-ad74-fafb832b24f9','e3973957-9062-4ad9-a568-6b1be3bd715e','b0b9dc3a-87af-4764-8e84-3675ae455abf','03ac423c-cf97-474e-bbf0-ebf6a6a518c7','d3689adf-d1eb-4ebb-a606-f0d59cec89e1','cd68ed29-2b99-4843-98aa-a83eaa8918c1','14048154-d915-41a5-bad4-5a1650878aca','bd8257d3-1875-42ab-a94f-6322f66d80db','7878ea70-fe8e-417d-9057-56f3afbc2105','9bf47cca-aaa1-4766-b025-2debe2ce73cb','87e1f1de-f0f2-407a-97e3-1b47be1d9dc6','d50e15ef-37db-406e-b4a8-6305cda53064','c552b945-6ca5-4280-b93d-57bc9c20c999','bd7917e5-6063-493b-a0a6-4d433fed06cc','7f37ab80-632f-42d3-aa4c-c6f5329666ac','1c5be7c6-2f94-49b5-bc5e-373c53f45f1e','cc5c89de-b2ec-4710-bc14-d97e3c18ba5b','d7050fd7-848f-4b07-9d14-11cf62bbab33','ed1eb5f5-2505-4e98-ad42-43520185341a','5943dd6f-efd0-4cdb-bc3b-ff3bffb600ef','76405743-6c3e-4692-b1c6-36a206be9d99','8f9874fd-1bfc-4637-acaf-8dee06e20089','0d2197a7-aafc-4543-a4d2-337c11d5b958','6697449e-3ed8-4e9d-b9d5-98cb84c130c2','71a07049-d6f6-455e-9066-6410805f4263','9e640530-fc8e-4998-9833-40b63c29fa94','8a26c2a6-6848-4a1a-8ac0-133415e2debb','ca557a0c-af04-4022-b093-c015b2fc8b3f','53e046d1-c7d0-4db3-a54f-11b65b001b14','d01030bf-c897-49ca-a746-6fc1591e9735','6769c3d7-ccb5-42c8-b92c-d6a11a8431e7','e0d0c01d-9883-4483-9058-925a40898471','2bcde915-8959-496b-8b1e-e0b6cd76eda8','93c5e67b-b342-44eb-81bc-4f43870b8ea8','a4a512c4-cf89-4337-bf74-389eca1eca3e','a04aad9e-3136-4f48-89ec-63e458c0b008','52a5294e-7e22-48c3-9160-e66b076eb851','8df6f9b5-3d61-42d9-8982-d6fc6bfe9747','672872d0-0aa7-4ae4-9410-0cb5f8877619','031fbbce-cd8f-4987-aa76-19e95cf6a415','e8341155-21d9-43dd-805d-b01b9bcddccb','6e594cf1-49b4-421e-9494-bb9db0a293f8','36db0792-c593-4304-99aa-8e3bdde889ca','bfd7b999-a88e-4ead-9655-648bea8e022d','727ec71f-c5be-41bb-ac92-0714b6967c2f','2a6d6e6f-0182-4bb4-8a35-a64b3587066a','05356cd5-96bc-474a-a16f-6ffc0246deff','fa962665-1110-4f7f-91b0-63e6df81a6f8','b15473ed-79ec-4fcf-92d7-f90fa8ab4eca','d2e4a8db-0219-4844-b469-df51e0d34a8e','5a6eac4f-a1ee-431e-9891-57969ecf8e35','b7cee7a8-ca8a-45bc-8c70-fb29e133fd37','3e0aa5ef-f53e-439c-ae49-1b5f65cdb852','973f6a9a-36e6-4ec4-a152-3eff0f53a33a','b0b7e9fa-4ba2-405f-b808-da329809d5fd','ad341250-1790-428a-a892-fc1101ed66c4','f0e895b2-ac63-48f9-814c-46a03cca0bc5','bf07cb96-73d2-4da8-8295-15c87fb1b59b','06de341e-d6cb-4e8a-ba91-9ab8a479b012','378afcf6-095b-431a-b01a-ab8d349bf953','79855f45-e2df-40da-8fa6-2cd6779199ed','e9bb2dec-c610-4cdf-919d-b4d7892b259a','fe5cce36-a881-44a9-af5b-d414768f65e4','399a6865-f161-4ad4-8166-87549cffed6e','a950012b-7639-4072-94a3-a5742c90ac32','e5ed0025-1c0f-4a9b-b995-840f176f6198','4e561e7c-e893-471c-9f78-604f3c7ce480','c69cc556-2f62-4ed3-a180-0117515c446d','efc33d76-1c4c-4e1d-ad6c-eb0f93dc49e0','6d018272-1ce1-4a57-9e49-32a2e6e3ab81','3e95bef7-258b-48f3-b1dd-1f04c6bcf098','4deca0e1-6412-4b72-a701-7aaa31f6f886','fed16c43-60d2-4cdd-a1b2-ab3d5d03b890','0c29aac7-f7e0-48c2-a818-1a410528d7c4','e1e26a52-7aa7-48ec-bdf4-292ae774d448','e686dd53-8f6c-485a-85db-188be9ad3254','1158d951-f01b-44f2-ae4f-c3aa5d46a926','59aa29c7-ff88-4f8c-aff4-135e7e705184','0d13410a-d3a5-4775-8b5e-8008bbd1d3e7','e0151ed7-3e5e-44fb-ab14-906a45b20c7d','754b30d9-0384-4843-af50-0f045246db6d','41bc20f1-7355-4670-a25e-fb26d8208c46','1793ce2d-ac64-4427-9175-64cb7ebba9ca','09cbb9a2-1a78-4cd3-a252-4c18c9fe74d5','01cd90d8-f691-46f3-9122-8a81a1d6f5d4','eef50ebf-77c9-4b31-b0d1-63d7bc1d49e1','3cc2a1f5-396a-4bef-87c0-2d737a7fa7b5','a6ea53cd-bc00-42c5-a7cc-6532ed6f5502','f327ce79-275b-42b4-8619-7f04a1fe2e58','05e66448-843d-42c9-8b75-8e7c732944e9','87c4149d-3af7-455c-9f88-2f27b5ab745a','80ce0756-c9e2-459e-8485-09a35021a7eb','162bd8f0-d660-4c9d-8514-72502384e446','917aaa59-51ef-4f53-8847-022d63076242','e379e204-b489-4c23-90b4-42ecd1bb354f','c012f383-559b-4b25-b8ed-63093f0c07b0','08ac3148-2b8f-4e2a-856a-0a814eda2de6','2684f6be-16d4-4ceb-bf18-a80b479e8afd','abb4bf4e-27a6-497b-84fd-cba742e586cc','490d6d4e-03e7-4bae-9d71-d4264bd600ee','a6cede5e-ef66-472c-af85-816813987fe4','13c30004-ae72-4b21-aa0a-127a28c526b4','ca7e4816-13e6-41ed-9054-6a4d977b2d73','b8c846c5-4fbe-4632-9062-ca420e2e6ffd','02793d21-64f6-4854-9ee1-37445e785e91','093f7ef7-ddb8-4a38-b39c-505b4c57aa2c','f2ad6940-d17b-4059-b6bb-cf29f35d43be','b5032eb1-8eb0-48b4-b231-9cc2c03b5c73','68fbddc0-025c-44bc-989c-0d4fb401ff2c','b9e735ff-c612-4a48-9562-5f7334eb1f45','57df5588-e871-4aa2-9992-58af5e5ec436','a7e002df-e41a-46ea-b29e-853045ef36d5','5193dce5-bea9-4285-a4b9-e20849f77351','d085bd4d-2015-4b9c-9e12-da7ade7e43db','2cf6f4f8-328e-42e7-bcf4-1580ebb88733','21420ecc-8b96-431d-a4a9-ab91f5714061','6ac9e9b4-e2a0-4418-9a0e-c857fd2785af','80ba12f2-e212-4ce0-9cd4-21ad91eaa1f3','5b875ee8-a4b5-403e-ac61-07e5e66fd915','1f3fece4-d4e9-4dd0-aa4e-8d67f3392797','51b24367-4fcb-4484-839e-52f095a435b4','e6cdc9e4-7d59-42de-8b46-ed09e0cf18ea','d5da61ac-5567-49f2-9381-2bb40c8feb72','78de623b-853c-4d32-96de-855e7a02469e','26fed6a1-5e3a-429e-8030-8a1cfea65653','3c205449-2844-452b-84c7-ea9d29d2824b','29a2699d-2ec5-4923-b4c5-876104574211','a1288ae3-4657-4b9c-83dc-84ede84d88cd','4a30f427-f750-4316-95e3-a136bbf62f24','bc725a05-7454-4086-93ca-c230da277995','fef6880e-9b53-4fe4-a38b-fecb9cc97bac','5ec9e8ce-dc57-4581-82dd-c789b347fba1','2fda9030-7b1e-42ac-b778-370855c00490','6ce5a03b-ca74-46ea-b8f8-312aaf708937','cd8d9989-bbbd-4caf-a080-31abd4cf95c6','a3d0436f-3b51-41b4-9bfc-0998bc864d23','2e82c745-6e58-441f-a3e8-14e9d47728d6','f7e72d74-36e1-45f2-aad4-3011e6878641','fa4935ee-7263-4529-8611-33156b6cd0f7','a00f6a69-e930-4c52-8ac5-d71f8c09df8b','a88bd410-4e1d-43c5-9ba0-a9ea1d182816','d3b5cd56-a769-4584-945e-015a91f9a184','c42d73bd-1a1a-4468-a2eb-640af80f10a9','0a0bf230-a3a5-4ffe-ac12-e4db2a71b475','b5d54455-e0d2-4384-b40e-d934996fffaa','9c16556f-fd62-445d-9eeb-947192dbc0fe','0b711082-4bc8-44ae-81f5-53600ba834a8','723f7bb2-dc22-4be2-855e-99a3b5688f54','483b5f5d-9b69-4543-9438-2f5174116275','e8dba571-e65f-4e82-b7f3-cf6be1188f90','b9a3a2b4-e155-4e5d-8c2a-9237c3b2fbff','66a64c53-b202-415c-827d-bd18947527d7','3227ac1c-aa88-4faa-85a5-7d09b760a648','3235541d-071d-453f-bb8a-d43dd1fd1991','deb3cc31-aa7a-47ac-b332-33185ab0066b','90e4ccf2-9fa7-409d-9de3-9cc21851ab40','8c47c83f-4256-42e8-9b9a-c626fff29142','900b06da-2457-486a-be04-d1f1432d1891','8647ef62-f711-4bc9-882e-45504cf841af','bcd97d52-f418-4f8d-8b77-d978f44d8bb8','a4c855b1-9c5c-4e6a-ac49-f597bfd80d92','ba355422-00eb-4377-a286-64ecb129340d','45ca6b5b-152f-467d-aac8-2d0b687d1785','7c969816-9ed0-4696-9240-32af54a2db0c','2f8f3f25-74e1-49ac-a2f2-e4af880a04aa','4539cb02-1d40-4dd9-b3ab-aac05e3df456','10c43e2a-03c6-4ec5-bf6d-d3b2e9dfad42','c8837f32-828a-4941-8d97-5a9fb9ff3f33','1b2f2680-4978-4bae-b84b-bd9d6cdaf323','3c8e77ce-a707-4de1-9e60-6a678f9fdb50','398f6fa1-5899-40b4-b016-0cd1b5677d44','52106216-4fac-4b37-b170-9d47b6af67a2','c01bdbb9-be1c-4a8b-9eae-523f9b2f022f','e49379b9-0013-4471-af45-29ac8a4a27ab','c75c2fbc-2206-4557-822b-7f43fdb2c62d','2ea42023-b2d4-4757-a684-40817d4e52aa','911f8cfa-ff16-41e6-b542-451be58d6d73','41421dcd-9c45-437d-b5ae-e804dc06e9c9','16bb36b5-7adc-4fb2-b715-bccd82b745f2','d7ad4b40-2783-4420-a4df-a20872943a70','1d59ddec-93c0-48f0-a777-ff025ea071b3','40b3dbcf-a7dd-417e-a29d-e3d856f21ef7','13f1f72c-8da7-41c2-82d2-3f9fa80bfa81','eb294fb3-1012-4476-8c72-d1cc0f6db464','973bea75-f19e-4500-a0d0-8f57158093e5','183259a0-2291-46b6-aad1-ba1abae36baa','75a4f547-39b0-416e-a0fe-90a29c016e58','95588098-9f6d-413f-9925-9c667a00ed69','7ccfaa7a-7367-4718-9374-9c9707a2a743','d33ce3da-2e8d-45ae-a706-51fc9b5960a7','c3a685c4-f1d8-4dd8-9888-6eb95e0f2624','8e944074-5a73-4255-8c7b-b01da9068e77','b9fbb88c-166d-4d47-801c-d57322f121e1','99ea22f5-a7c0-4fe3-8506-3463282db86a','67b32cb7-0392-4dfd-8fe0-95461ef59cb8','62091544-a674-4539-9f85-66b5fe868edc','0871086e-28df-408c-b024-79a4807fd8ef','4e41aa96-7567-49c5-b177-a1eaef03ab88','9a15ccd8-d0d7-43fa-8a25-f9f80a06c794','3101a422-5c47-4b93-a682-2615a26058c6','24c54d17-dcc7-4686-81eb-8aaa6f515099','e382c535-4dcf-40d1-909b-c8d3de674f3f','1c55ac28-7ef8-4341-883d-4e6501d117d7','a4df3709-42bb-4f2a-a454-bbf8466feee1','220271ca-db81-4242-b750-4a1612ed94cb','9c274ca3-309d-4504-b88d-ffc608d60a1b','1722b31f-e93b-49fc-9648-0886073bfeae','08b78d57-236f-4785-b4e6-5af03be5a13f','34a8bb60-ad67-4dbe-9456-4660d6a0aafe','acc85fa2-69c3-4b8a-a489-f564690b1612','e7383133-7029-4d30-9c2f-e1ac0b85a1fe','9be4c5ee-97e0-4225-85f1-57c6ad10906b','c4e38de8-167f-4772-8bee-e16e5224d5c8','e4eddc71-6999-4e12-9da9-194b87634f4c','2632274f-c67f-4533-aff4-67b685dd5a0d','882b4fda-4138-4458-b790-eafd6920cd2c','81f3f756-5a1a-4235-aa5e-27cb44054c76','660116fc-0b5e-4844-8151-5740611c85e7','7a1acb56-bfbf-4f52-9de5-139a2ff9aa3b','8742b360-aa47-4fad-b8b1-28385ec9403a','f6081493-e330-41d7-86a2-414a4205506a','8b083e32-87aa-4a42-936f-8483cba296f5','8e832079-56b1-4b34-a2ff-c6ba5e4a3df5','49c7ea73-350c-44a7-ae50-0ddde66359dc','294fd3da-51ee-4ea0-b56b-4921ded8e16f','af5bb021-46e8-479a-8cb3-0ead4957ae02','851c37b6-f96f-4e8f-bb92-2e2a6213f45d','52e42139-3573-4af5-bec2-e06e11353b43','c5fbcf1e-9046-424a-99e2-345055e64424','dd03b6c4-706e-4c1a-ba54-81f12d9fc552','f1e02b67-22eb-4740-a4e6-f9c8a2e49dfd','1261f927-6f2d-44d1-b11c-e1df8070fbf1','564465fb-c220-4e00-b2a0-d118e9034944','90b311eb-3975-4e3d-a48b-d9177245faa8','996530fc-1de2-4e8a-860d-1ec198940f86','06084a1b-0e01-430e-8001-68ed0590183c','d9f7488b-5636-40cc-bc87-b53c6c2e3d08','0a6eccb2-e818-49fd-bf7d-c7d3f6c886fc','86847077-6d78-48af-a31b-ced456dbe9a5','30a7ee42-b875-4d95-8af9-ba7e2cebaec5','262deb12-1140-4693-a3c9-2c15e432a8ba','7c2be1ab-3379-4e2f-9ec8-dfcf2e410a4b','6af0dfc3-2856-4a65-94ac-730d4defae37','546f6022-2599-4580-aa7b-204507963f39','efaec79c-1039-42fe-b6b3-5f34b0e95e9a','f1de6261-98b4-4d6e-ba05-aca3b990205a','ceb1c758-ce03-4ce7-846f-64ed1e80f5e3','7406c181-30b8-48e9-924e-19367a91ab68','9058edcd-72a4-4bbf-acd1-3db6efcf715d','5a41a3c5-867e-4476-8bc2-000fe6403130','67beaea8-9328-4ad5-9c12-fed2fae3caa2','6e8f900b-8776-4784-a934-8e7638a46631','9e352614-d4cf-4469-abc0-bba2a3463117','65450acd-ce8e-40d4-934a-90d1c1f56f34','f4c47e8f-1c91-4181-8601-398f02c1cd5f','ef93f398-a779-41bf-9643-181212a6b65b','a512d60f-7954-4d78-9948-d63769261420','47ec82b9-be54-4007-ab5c-61f48079b175','59f95816-b3ec-4006-96ef-24ed4ddbacee','696d1faa-ff56-4c1f-886a-43cd2808243b','96f12253-25d6-4ae4-a51c-c3a2e797e489','4830a93b-cbaf-4f99-ac45-b63af4204b97','ea84d1bb-3fca-4990-8ac9-edd76ef95135','c43f1500-fc8c-430e-b3cb-680ed23403eb','d94ad5af-7aeb-4bd3-8a48-70bdc5a6bbbb','10fb69b5-8f52-4ac5-9c6e-0e3173a12d9e','f2ef88f1-6ad5-49ca-a08d-43abd9886667','e004f25d-3aa4-463e-9583-901b2d6a6d6a','7b699cbb-f399-4305-bf46-19023e92f9c8','df7e823d-2243-471e-b090-72fbfff62481','b3cda696-8fbf-4dbb-8ee3-4f52b91f8215','f7714904-f458-43b5-b7b9-f56c8bf971a7','adb2f5b7-7229-44ee-b8b6-7acdb43bc19d','abee3455-64b1-4eb8-b982-e6ab9039bdb2','72f7867f-529c-4afa-b1dd-c4b86b928914','657f3805-d20f-4991-a246-1391a2ec4051','512d77fd-011d-4550-af9c-6a379f69c476','23fff749-a440-4bbc-a659-af768fc5fa11','dc7536f0-1823-459c-83f6-a5e208acdd1b','0704a7a4-e47a-4b4a-a284-86f114bc389e','1a0d9703-d925-4862-8c5b-9895ff1b7a5c','83154dd6-f530-447c-a146-3daf61e87f43','c5eb5868-9c2a-4bb6-9b55-014b1e2680d6','326f066f-c5b9-44df-802f-8f86ca15d524','18e4f248-bf17-4ee3-b826-c7bc2b69a016','4e5877d0-3a96-464e-8e82-1c74cbe0de98','9d373d47-87ed-44d7-936a-201575d77e71','a3ab1744-8d0a-4d5f-9a1c-0ba826744726','73a30c95-a6c6-4588-b362-a911bc5d9f6f','de350dc5-895f-4455-a023-fcbe97cac6de','595cf701-59d8-4987-a38c-c3a2739a5778','bf01667a-878f-4fc3-a0cf-ae8a451a74f1','e9199c9b-f48b-42eb-adba-13f3dd50aec1','e0510624-e397-4423-a402-ec9781263ee0','d27cc41a-45ff-4ce1-a1aa-97018901586e','eb730d50-7ff2-4bf0-ae62-7988602ddf8f','cbfeb3a0-a2cb-4897-a099-52c579c14342','1947247e-89e3-42a4-924c-5f13861f217b','36f339e8-58ab-460f-8ecd-776ccdc9ac51','f5c0e0bb-c99e-4e95-bdb6-69111f5b1b68','a2ca2edc-b970-4466-a4b7-cbb0cda6b53b','bf248c25-bb7c-407e-90a2-41508bd8437a','31bdce24-a5b8-4ebb-a944-e94d6039c848','d376c50e-2071-4498-9146-9b3eb4e0b488','36316b21-64a0-424f-bcbf-d3d095461fc9','78da13d6-73fc-48a6-aa5c-b6e0149ab21e','8a0ed333-b1dd-4ad2-922f-f31939d1f4ec','ba42e23f-ab34-4665-9a96-251a98b3123f','562781ae-a1ac-47bf-a498-3250f97bf143','84c79bbc-9d04-49dd-ad6a-e288a0419e61','8c8da157-77df-4fc8-a172-33f115f82d86','d8938378-c80d-4eb1-995f-fc29c78b1bcf','9e39b1d1-c3c1-411e-982c-bf576f5285dd','1af8ed30-8e8d-474b-ba38-4904512991c8','f891cc29-1d5f-4869-87b1-29b7974b55fb','9c9bc5b8-d193-4cae-a0f6-94cf3a74eb8c','01bda7ad-17c8-4423-a77d-5f0c8caaba70','4703bece-0442-4573-92df-6eb8a33d8cf8','b616b8fa-9b9e-42ff-a6a4-0a2805e2a95d','95dafe46-85ad-42ba-b362-a2738ccf7cee','e81de25f-52bd-474f-a5d5-f53b4f4582a2','bdde9640-8679-46b3-bc18-5121037c83a2','711093b4-499c-42f9-8cbb-18ee43381bad','a517b8f3-bd5d-4227-a447-ea3305e2bb07','56d4c00e-48d5-4298-88e0-9701049f3f23','0dc9458b-9c87-41a1-a971-ab6747403ab7','fc8a518e-24a8-4224-b693-6ef943b6afa0','bfe2913a-1c3d-4c19-9c8b-6a60c52f65f2','b10459bf-aed1-49e0-9134-28fefe604917','d0af9589-d05f-49a6-bbe7-c951d9c2909a','b32c8235-1bff-42fe-b256-37ac73a66a39','c7aa4c37-f938-4f89-b7bd-9fd3aa47a8f7','a2408b83-d230-426b-9ce7-6bf505469410','a1c63f60-f891-4753-b6e5-c201a412f0ee','19ee631a-6273-4dfa-9704-57fbe7351d57','38daf67b-c4b9-4c13-be67-bc158d3b8655','9775c866-06db-443b-83f0-5b386e2f8d00','5f72c826-399d-4d1a-9542-5a45a7635b85','cebb9bb5-87fa-46a0-ab62-1f3d653ad4d1','bc91135b-ad9b-4d30-9c88-dbd7f2136da1','1644bd18-28e3-4894-b442-9874fd3c59ef','126de5c2-6b77-48f7-92b3-83f907d3e6a4','52c471f2-477d-4d74-b267-4fc22c71546f','f4ee96f4-7fd8-459f-9d37-d6e1fdbec284','6091d34c-8f0d-4e40-b10f-772e7b26a826','43a701f5-5603-46f0-a388-63d482fc157a','3c63ba95-67ae-44c5-a058-6f8f7ec286af','3eb4a871-28fd-4ff2-8372-e1dc8c8b891e','96fd54da-70fa-432b-a4e5-d85f2363b12f','3b706f7a-0522-480e-be62-1c08ef89040b','bb109726-f71f-4d38-a4f2-ad9d6ae36209','29a491c7-a1a1-41bf-b813-345dcb8fcea2','3d4b673b-a431-43a7-98d6-91e1a1ce9d12','f255b9ee-82f3-4083-aac0-cd47d2f133c7','36f056de-ef0e-4c44-aa9f-35e8797a38c7','af245fa6-7ee4-4309-a228-a37460d1e3c0','ba5074ff-e999-4a73-8e3e-b76ebba07f20','821b004a-785f-48ce-922b-19032ba425ff','9ccfed79-dda2-4022-a92f-34df54d0eb24','e432cad4-68bb-4dcb-a550-ae13e353ef89','32557973-9d50-47e2-88e2-f21511d5ccb9','73de089a-32e6-4321-a971-b3b795141ea8','46b6b524-b8f4-4f70-846f-0e5a3154f9e0','5af1299e-cca3-4be4-8b40-eeefcbff7cbd','5b15bae7-ac75-49aa-b373-d82855f6af5d','f9164112-9f30-416c-b709-946e5381e24f','575373e5-513a-4309-bead-7ee3f854cc1a','7df7f977-b65f-4971-8b31-8da304c59274','ac329982-edef-4ac2-8e21-a1b295d29c46','d672d24f-0f4b-4b36-b506-7d002c8603f0','7c8a7889-d2b3-40a5-a19d-ca2600b3e308'}}),'800720',struct('BlockId','c80a3eeb-3068-4a29-898d-f741620abd96','SignalIds',{{'792751bf-2cd9-4b9e-9e6d-dd8477eeff11','fb3ae2a4-9350-4dcb-9791-bbe9a2394ee9','a07fba04-c60c-4873-905d-c8747c4feea5','37a2b510-37bf-466e-b9b2-1bc26afdfe38','7fca05a8-dc01-41ed-a206-a11d6be68458','ef3a0af1-8e41-4e57-8abf-befe27c2e93d','88f73851-6028-437d-a26c-7a024f907c6b','f0d2dc69-330c-4035-b933-fb80c16e0053','f75b582c-d499-4b97-b6e2-5aeaced233a2','0b656d8f-e77f-445a-b9cb-efe4cd684130','73ed5008-8924-4395-a20f-7dcf83ccff51','b42e8d0a-b18d-4c52-9c0a-3a5f2baaaaa3','817e5c95-0703-428b-a5a6-7ff306c04c72','fdc89135-b01a-42d6-81b9-4abf1d9cf4a7','ed25710c-9946-464b-b719-c8dec04fe409','37ae28a9-ab21-4c2b-9685-b01ecb5f6107','45c9bb8d-1659-4863-a8d3-46a32c92fa2c','f25d56f4-64fd-47a6-9dc7-f211f6269ca1','adfcb8af-eddf-4798-af01-dc0f8438d67a','387368be-8cd3-4c31-9a01-474e7adb8391','1d04f81b-736c-4e73-93b3-7098fe3582bb','4dc4d9cf-dbdc-4bbc-b917-75dd652485ab','b0247cf5-17df-44fe-8485-89fdea12044f','cd810d09-56e9-47e7-a012-f593982800c8','83e9a486-4b80-4875-8087-190cd09e5bcd','181ebea1-b178-4b8b-a500-306716504ff3','ef21d6a5-c94c-42be-a2f0-f7155269a102','04d11ff3-28cd-456d-9ff7-e602b0edd237','17844e58-beb0-49c8-b33c-538e64bc86e9','59152c6e-2288-421e-8233-5bbb159e7c47','15898122-ff0b-4a4c-8b5c-85a17514d3e2','cc4d960e-8cb2-4ac2-845d-57424825b1d7','fe5b6b5b-31ed-44df-9ec2-3ade09078e96','4a6a8c38-8696-4162-8d29-1795e715c650','f4a87070-2c88-44c3-9726-b1d2d6dc8569','c61715a5-101d-4a9b-b9c5-e3ef6acfac80','635776df-9ff1-4017-9be8-9f56ba364905','8c4e4a86-8be1-4361-b471-e235e5354897','9b7961ea-23ba-43fb-ae3a-23e1c6a0f712','bb7eed17-780e-4281-a07f-8b55579f2c66','b7afbc56-c91b-457d-8806-93b72870782d','1b904d85-91c3-4ab4-b5f0-3600587ee8f8','0662a30b-5d43-4d34-a192-597966fbcb33','bbb6bf05-d916-4ea2-bc2e-819bd54b717f','7a8cb35b-1475-43cc-8f53-78d1bdd2f4d0','377a87b6-47b0-44d6-a78c-35c68aad793d','e983537a-ac5f-4f4c-9f76-31f5d44baae5','de0c751d-fb24-40f7-828b-92ccabe68ef3','fc84022f-5f43-4507-934b-a6a35cb8e772','cafee757-34a4-40d0-a0f1-063f72d448af','aa348eb7-37f1-4f94-a261-9f557ad63a17','3ea7c60b-7297-4293-ada0-4c38e0e184ea','fb235619-8741-4030-8cbb-2d4e0c052574','8a2113bd-9c01-43a6-b56c-0878a8cd316d','128237be-1d89-4f0e-973f-8f86c711e76a','e887201c-6e5f-4390-981d-0f72cf6bb427','850f4906-068f-44c7-a0ab-313ec930887f','021ec8e2-8cff-4adc-bfc3-0a9c3497ea7d','544e4ecc-afa0-4b41-958f-6a4d5bc840e4','92c2544c-13e0-4d10-9e48-50681df4870c','76bf4179-8b24-4ea0-aebd-ead989d2abdc','455b0e82-5064-4a00-840c-8a29d463eae7','3ef9da80-1855-4d84-934e-cdc409abf96a','0e2ba2d2-2712-428f-96f0-4bccc97a26ee','3508f21e-abdb-45d8-8c9d-a455e46ddab7','6c4d96b3-7e22-403b-b955-203d6ca9a45d','48d07e43-4ef7-4d37-96a2-baeaaa3d188c','af0193bf-3936-492f-b6a6-52e6d91ab91f','8d36bb1d-cdd7-4cbb-831d-9439621d9016','d9273391-7fda-4d77-9d07-13e604f9df4a','f7c128ae-6cfb-4a00-8c26-01c934c937cc','a218ba25-d127-42d0-9318-2c761c88326c','7ef79124-cd50-49a1-b905-4d40bb38361b','414c2708-f715-4eb3-bae1-dbada25e0484','f262efd9-ce0a-4847-a01b-48456e77c9fd','cca526f5-6aca-4739-b408-8079914ec954','e0fecd4b-8638-4f3e-9dcc-57c69bf252a4','67e9d417-3570-44df-b72c-254913aedb50','76bf18b7-59cc-4bc8-a5b2-a6266ef9e8e8','20272d22-c77c-4c76-b0ee-44150fc9dae6','7526ea31-78e1-470c-9b78-fdd078e759a6','3d2abd71-adfd-4079-b986-82d9041e7dee','2f99155e-5a4e-400b-a298-99c59b2836e4','0d7c66d5-d8d4-465d-a089-9d3b5c6750a7','bc53506e-24a6-4c83-8919-16950f3d9e78','8747e9ea-5dc1-4e44-8205-a656959defcb','afb9a0a4-e664-4bb8-9bf7-42be658241fd','2b92f684-e9b4-42b5-90ce-9498b99ca146','8c1a9f70-e041-4f5d-b720-b33d0c5eacbe','a090aa33-a2b9-4615-b630-9877b87eeec9','1a7a46c3-547e-4a1b-93c4-6c11472ed80d','61150f6f-0fd7-485b-962a-31e5b0373fd3','88d634b1-2b76-4f3b-aef0-75b29cd76362','979b189b-d29d-40e2-98c3-487408080559','bef4e043-9f63-4bc0-9aff-d0c9430d1f84','aa48750e-3eeb-4d95-b1e7-d6843bd81d51','76f35383-fc5c-4f82-86b8-bb9bf3022dca','7d659b64-42cd-4107-afc3-168f727def97','5324f823-cd4b-4c55-a0a8-2f30f5b651a1','4a23a02a-c4c1-4811-bacb-4669be1d7a78','6594d32f-0c93-436c-972c-b4d4111dc09d','208511d0-43d2-4803-87de-2daee199bd89','b1802160-9338-4883-ad05-ae087293ecc5','6ac2cdf8-ca88-4f0e-96bb-ea532280bbd0','01f6b648-349c-4695-bd57-c7800d390439','b125330a-88af-4ef2-8836-c4b90a82eaad','16568bf3-237c-49a0-98ef-9f74e6cb4366','951ee8fc-d618-493c-86ec-a45f134d6a9e','f662f000-80fd-4e61-af98-37cf73da68aa','7e57e338-50d3-427d-abe3-82fb00cde3cd','c8ec0ac8-8dd0-400b-9bc4-3d6a4259c7d0','d474232c-ba79-4b0e-8f01-7c85907ec306','d23c49df-81d5-4b57-a158-28d81834fac7','011e468e-b123-4e6f-a478-1e54de974d05','89f4ec27-9e61-46d0-a50c-e5fad8b7a200','baac12cc-ebe2-4eb8-8c44-a4252bfe1813','2f8ab832-d1d6-4761-a743-28b5ad4317f6','27c5ec8b-72c0-4692-bc7d-352ecb95cda5','716f7a17-0a09-43eb-afe3-0dc18b58f39b','267fa3ee-6491-429a-b5ab-ef8ac89f168d','a64113d9-dd3f-47be-977f-0f44fb2a71f1','14a94e30-e317-4563-87cb-959d64f06af6','2b2451b3-90a6-4a5d-93a3-7a226f90a1a9','f3d32815-fb57-4d56-9ff2-971c89dc90c0','33e4a5b5-337d-466b-ae02-8a59bb247cdf','380a1646-2df1-4d72-94cc-f5c321a813ca','60326851-cf17-4258-8572-d9b84952a8b2','619116f7-7bfa-498d-93aa-bb6ab5822816','afc30dde-4125-4c61-aef9-20d3088f4870','dddf9368-52e7-4fba-9af0-926125b8c4d8','c55164ba-f16d-4407-bdad-50bd0b0d9f7a','bf0a35ad-98a2-4511-a385-10930f0d108f','f235497a-90d9-4dc4-955b-9fdd922aadbd','4dda3e91-c19f-4eb5-933d-2193cdfe756d','9e6db103-952e-4e2a-b44d-f73a9357be99','3dc9ddbb-83cb-4e83-bb6d-2dc87b38f224','05c7ecac-01dd-441d-af78-9bfd2f469f7d','3e25fef9-2ab6-4693-824e-7c48e669ea59','bacb3a65-13cc-4e3b-88ce-3a5ab2dcd868','330cc210-1b52-47fc-8bdd-7c1a4b18bb63','dd7055ca-fd93-46f8-b41d-8ae87826c4ae','752798da-4900-4f43-97d9-ccf189742905','8bf4899a-edcc-4a5f-a228-4ffb7cb4dd55','2f5a4419-d17b-45a0-a008-6c4523297653','fd4aa567-1940-4011-a362-e6944c5cdcec','90a971de-089d-4492-a05c-1f0baacb1fdd','43b0479d-10a5-4376-9ad3-b002165e1a80','001fb65c-cc6f-4fc2-baea-b774086eae2b','01d7fe59-23c7-432d-b552-117afe645963','e438ea04-c79c-4de0-83f8-b502d5ddc513','cd08021d-974f-4dbf-976e-e6b3ebf6c2da','fffaf1ee-b98a-4abe-917d-8d3ebe971afb','1dd87df6-b509-4616-8f1e-1e84fc6e89c9','48933dde-bccb-4a7a-8dab-6d79e00794d0','1fc3471e-dbcd-455b-a2a2-6192cc95198d','ce55165c-1498-4331-bd1e-b92210708138','1804c5ed-a1b3-49dd-bfa2-3e47939f6ea0','52d25e9a-df63-49ee-bdb8-9e6a75af42ec','04e0fce9-c5b8-4eae-9d3c-793a7aa01907','31e21525-e02f-47eb-9551-bbcc4b411747','968786e2-f1e1-4cf8-9c54-b7a23396bc2e','e3bf4a9e-eff8-41f7-b9ec-8238219ac767','3e8bd276-8666-41f5-a5a1-df6c08149b36','55b473c9-7fa1-4561-8831-e3fae4f313da','6836bfa6-bf2a-4a97-be12-4aaf7d996716','b7960b48-8164-46b7-9dcf-056550ad1840','3ba5441b-cbc0-45db-bdb2-cbcfc1404bc3'}}),'800721',struct('BlockId','bb4a0ad3-58fc-48a3-b23a-0496edcddc68','SignalIds',{{'8ebd732e-e5ed-4598-aa5f-aeda63bf5182','29d02400-ee1e-464c-b585-3e06b7107501','14e9fc79-6817-4848-a24f-a3abcaf54c43','f76b9df9-cfc6-4106-8025-1d261f15d404','c3afc08b-5447-45a2-8b79-854c28bcc6c1','1ba64e05-bb5c-4d68-a02d-9ffb02686de0','86122933-ac36-4aaf-9113-2887600b994e','f035a19f-500f-4b21-bd71-983f3236dab1'}}),'800722',struct('BlockId','dbbb41d6-bca5-443c-8695-7618582e4bf7','SignalIds',{{'a0e6bbf9-a1fd-403b-ade1-e47ba42e06b5','7c8037b0-4d3c-4c38-94de-7493ac012a47','a2e41dae-6b49-4c2c-956a-b778509fac85'}}),'800723',struct('BlockId','1d124506-3787-45cf-865e-b4a57d238a51','SignalIds',{{'0d0a6df7-7811-4a6c-871d-5b47671a7c1e','721bb71b-22a0-48d0-944b-27ecf9853cb8','ac147e37-0c9e-4fe6-8c66-980dbf93356c','8d77690c-586c-44aa-8e86-1ddffb4dea32','26cb938e-39ab-41ca-a420-281f820fdb4e','8fe97dbd-14db-471f-9637-80afc4e5b46d','841b8cc2-5b8b-45c9-a4f0-8f49ed75a59d','fb7447da-d48c-470a-b836-191daf3f610b'}}),'800724',struct('BlockId','402394e4-b8a4-4d88-81e1-4266c36d4e48','SignalIds',{{'88ec0713-91a3-461b-8d70-b7589519652a','0a262528-dcfd-43df-a8a2-e404b744fd18','af691278-8d5b-481f-8550-144157f31189','c414c8bf-cdb3-4c9a-9dcb-e75ee0e02dc4','43a7017f-969b-412d-8a09-7057152f1366','55e8f277-4804-4492-a829-4335b5f0b225','849d3a69-45d8-4ac3-a72f-d24f53a08578','042365e5-f4b8-4454-97b1-3a9083c3a898','48e11817-df79-486a-bb3f-ed3b2664aa54','e2669b25-56eb-495a-9b7f-773d7f88a887','d4dbc5f0-bc69-413e-b9da-25f0a15baccb','77a0940a-cb44-4363-8177-c699d8264a77','a484db10-7cb9-41f3-b70d-58f475a0796d','ca23f209-e1a5-4f12-924e-252646ce5130','9aad5633-cff5-4c45-9d76-4ef292aabef2','d54a7b1e-4326-49a6-a385-cf1a07279e5a','d018fa4e-06c9-4231-bdc9-c40698ff4fb5','420f4490-278f-47c7-bbe1-572bf33d0764','ebfdff75-a7dc-47ed-bfbc-131b5be4d898','20486cef-92e6-4c2f-96e9-cbafbd51d65c','2c204fa4-5680-47f0-99be-7a3b75ea476e','dd5739c2-2379-458a-83f6-fe0cdec450bb'}}),'800725',struct('BlockId','2d1438ec-af83-4503-b922-f47341c9b178','SignalIds',{{'6491420f-69d5-4244-a0d4-d0ed9ac132e6'}}),'800726',struct('BlockId','3d418214-fa71-448f-b039-3b1a635abb5e','SignalIds',{{'346dff9b-f581-4c3f-a767-f0ec0fca0ef7','efc1d03f-b7b1-49bd-92f4-6d0f1e28c751'}}),'800727',struct('BlockId','5e296976-60f1-42f5-b886-c00fdae99a6c','SignalIds',{{'0458605c-3525-41b3-9adf-54baec750c72','f3d92ea8-f533-4cf5-9027-9b22fb3523b1'}}),'800728',struct('BlockId','dceb43e2-35c8-4627-959d-3dcb894cf346','SignalIds',{{'b70ae306-1491-490b-af2f-6ad7ae877354','2b5ef35f-1fb5-4484-8472-8381f3f7e375'}}),'801193',struct('BlockId','0691fedf-9a26-411e-9205-0816e9e8cdaf','SignalIds',{{'d235ca88-6e86-4545-a3db-d3e1c5824f58','3a9384ab-4a5c-4127-bf98-74cdc576e344'}}),'801194',struct('BlockId','391af5cd-2ab0-4166-a8d0-49aad02fb215','SignalIds',{{'52fba00e-47f3-4dbe-b043-605b696bb030'}}),'801195',struct('BlockId','7b19df32-c236-4470-8bfc-3eddf1e643d8','SignalIds',{{'8ac81b03-a61b-44ab-b979-f2af65f4fe30'}}),'801196',struct('BlockId','712532a2-f3ab-4878-b158-f2db2062076a','SignalIds',{{'191257f6-7618-4dba-8fe0-0811922de77e','83b04bdb-8491-4cc7-a073-a4374c3e2792'}})}  ExtModeArmWhenConnect=off  Creator=dSPACE GmbH  LastModifiedBy=bxr240009
settings DataIOCC: SaveFormat=Structure  SignalLoggingSaveFormat=ModelDataLogs  SignalLoggingName=sigsOut
settings OptimizationCC: BooleanDataType=off  ConditionallyExecuteInputs=off  OptimizeBlockIOStorage=off  BufferReuse=off  GlobalBufferReuse=off  ExpressionFolding=off  LocalBlockOutputs=off  InitFltsAndDblsToZero=on  OptimizeDataStoreBuffers=off  BusAssignmentInplaceUpdate=off
settings DebuggingCC: SignalInfNanChecking=warning  SaveWithParameterizedLinksMsg=none  MultiTaskDSMMsg=warning  MultiTaskCondExecSysMsg=none  MultiTaskRateTransMsg=warning  TasksWithSamePriorityMsg=none  CheckMatrixSingularityMsg=warning  PregeneratedLibrarySubsystemCodeDiagnostic=none  StrictBusMsg=ErrorOnBusTreatedAsVector  NonBusSignalsTreatedAsBus=error
settings HardwareCC: ProdLargestAtomicInteger=Integer  ProdHWDeviceType=Custom Processor->Custom  TargetIntDivRoundTo=Zero  TargetEndianess=LittleEndian  TargetHWDeviceType=Custom Processor->Custom
settings ModelReferenceCC: EnableParallelModelReferenceBuilds=on
settings RTWCC: SystemTargetFile=dsrt.tlc  GenCodeOnly=on  TemplateMakefile=dsrt_default_tmf  RTWVerbose=off  RetainRTWFile=on  Description=dSPACE Target DSRT - Generates SIC files for import by ConfigurationDesk and VEOS. Provides code generation for Simulink models imported in ConfigurationDesk.
settings RTWCC: CustomInclude=|
  | C:/Users/bxr240009/Downloads/bim/real-time-performance-analysis/dependencies/acados-v054/buildVEOS/install/include
  | C:/Users/bxr240009/Downloads/bim/real-time-performance-analysis/dependencies/acados-v054/buildVEOS/install/include/blasfeo/include
  | C:/Users/bxr240009/Downloads/bim/real-time-performance-analysis/dependencies/acados-v054/buildVEOS/install/include/hpipm/include
settings RTWCC: CustomSource=|
  | "C:/Users/bxr240009/Downloads/bim/real-time-performance-analysis/build/desktop/controller/c_generated_code/acados_sim_solver_ecu_vehicle_nmpc.c"
  | "C:/Users/bxr240009/Downloads/bim/real-time-performance-analysis/build/desktop/controller/c_generated_code/acados_solver_ecu_vehicle_nmpc.c"
  | "C:/Users/bxr240009/Downloads/bim/real-time-performance-analysis/build/desktop/controller/c_generated_code/ecu_vehicle_nmpc_constraints/ecu_vehicle_nmpc_constr_h_0_fun.c"
  | "C:/Users/bxr240009/Downloads/bim/real-time-performance-analysis/build/desktop/controller/c_generated_code/ecu_vehicle_nmpc_constraints/ecu_vehicle_nmpc_constr_h_0_fun_jac_uxt_zt.c"
  | "C:/Users/bxr240009/Downloads/bim/real-time-performance-analysis/build/desktop/controller/c_generated_code/ecu_vehicle_nmpc_constraints/ecu_vehicle_nmpc_constr_h_fun.c"
  | "C:/Users/bxr240009/Downloads/bim/real-time-performance-analysis/build/desktop/controller/c_generated_code/ecu_vehicle_nmpc_constraints/ecu_vehicle_nmpc_constr_h_fun_jac_uxt_zt.c"
  | "C:/Users/bxr240009/Downloads/bim/real-time-performance-analysis/build/desktop/controller/c_generated_code/ecu_vehicle_nmpc_cost/ecu_vehicle_nmpc_cost_y_0_fun.c"
  | "C:/Users/bxr240009/Downloads/bim/real-time-performance-analysis/build/desktop/controller/c_generated_code/ecu_vehicle_nmpc_cost/ecu_vehicle_nmpc_cost_y_0_fun_jac_ut_xt.c"
  | "C:/Users/bxr240009/Downloads/bim/real-time-performance-analysis/build/desktop/controller/c_generated_code/ecu_vehicle_nmpc_cost/ecu_vehicle_nmpc_cost_y_e_fun.c"
  | "C:/Users/bxr240009/Downloads/bim/real-time-performance-analysis/build/desktop/controller/c_generated_code/ecu_vehicle_nmpc_cost/ecu_vehicle_nmpc_cost_y_e_fun_jac_ut_xt.c"
  | "C:/Users/bxr240009/Downloads/bim/real-time-performance-analysis/build/desktop/controller/c_generated_code/ecu_vehicle_nmpc_cost/ecu_vehicle_nmpc_cost_y_fun.c"
  | "C:/Users/bxr240009/Downloads/bim/real-time-performance-analysis/build/desktop/controller/c_generated_code/ecu_vehicle_nmpc_cost/ecu_vehicle_nmpc_cost_y_fun_jac_ut_xt.c"
  | "C:/Users/bxr240009/Downloads/bim/real-time-performance-analysis/build/desktop/controller/c_generated_code/ecu_vehicle_nmpc_model/ecu_vehicle_nmpc_expl_ode_fun.c"
  | "C:/Users/bxr240009/Downloads/bim/real-time-performance-analysis/build/desktop/controller/c_generated_code/ecu_vehicle_nmpc_model/ecu_vehicle_nmpc_expl_vde_adj.c"
  | "C:/Users/bxr240009/Downloads/bim/real-time-performance-analysis/build/desktop/controller/c_generated_code/ecu_vehicle_nmpc_model/ecu_vehicle_nmpc_expl_vde_forw.c"
settings RTWCC: CustomLibrary=|
  | C:/Users/bxr240009/Downloads/bim/real-time-performance-analysis/dependencies/acados-v054/buildVEOS/install/lib/acados.lib
  | C:/Users/bxr240009/Downloads/bim/real-time-performance-analysis/dependencies/acados-v054/buildVEOS/install/lib/hpipm.lib
  | C:/Users/bxr240009/Downloads/bim/real-time-performance-analysis/dependencies/acados-v054/buildVEOS/install/lib/blasfeo.lib
settings STFCustomTargetCC: SystemTargetFile=dsrt.tlc  MultiwordLength=2048.0  ParMdlRefBuildCompliant=on  GRTInterface=off  DSTargetArchitecture=32-bit  TRCGenerateLabels=off  TRCOnlyGlobals=off  VDFType=TRC  TRCGenerateParamValues=off  TRCGenerateDerivatives=off  TRCGenerateStates=off  TRCIsOmitVdOn=on  TRCGenerateVirtualBlocks=off
settings GRTTargetCC: CompOptLevelCompliant=off  ConcurrentExecutionCompliant=off  CombineOutputUpdateFcns=off  MatFileLogging=off  CPPClassGenCompliant=off

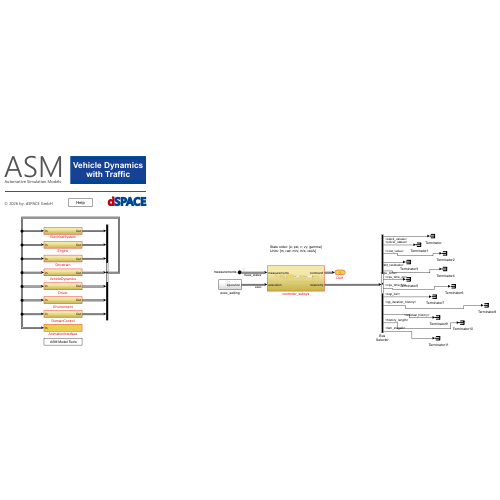
[thumbnail: Simulink's stored preview of the top-level diagram]
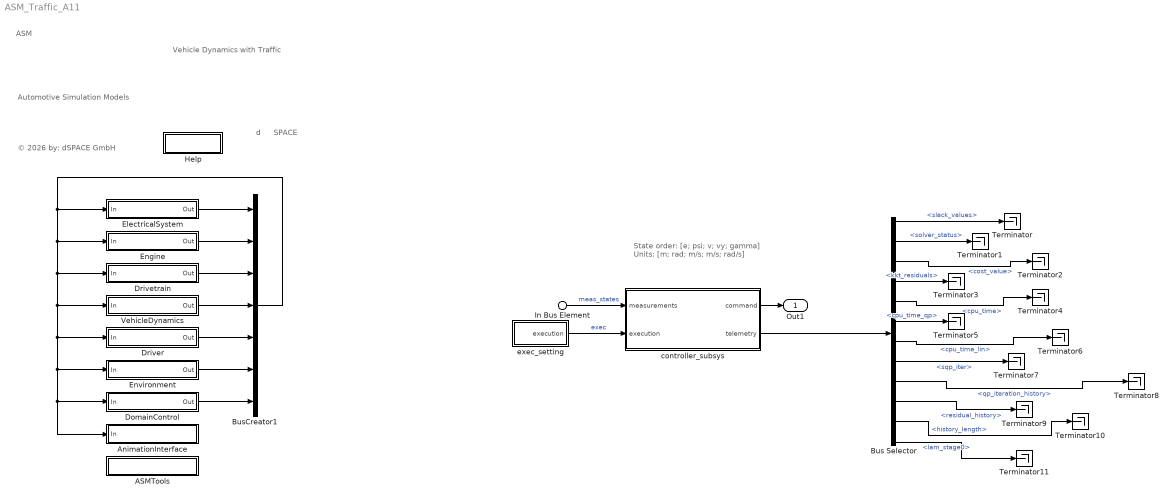
== system ASM_Traffic_A11 ==
  note: Vehicle Dynamics with Traffic
  note: ASM
  note: Automotive Simulation Models
  note: d
  note: SPACE
  note: © 2026 by: dSPACE GmbH
  note: State order: [e; psi; v; vy; gamma]
      | Units: [m; rad; m/s; m/s; rad/s]
  In Bus Element : Inport  PortName=measurements
  ASMTools : Subsystem
      mask Display: disp(' ASM Model Tools')
  AnimationInterface : Subsystem  Tag=AnimationInterface
  Bus Selector : BusSelector  OutputSignals=slack_values,solver_status,cost_value,kkt_residuals,cpu_time,cpu_time_qp,cpu_time_lin,sqp_iter,qp_iteration_history,residual_history,history_length,lam_stage0
  BusCreator1 : BusCreator  Inputs=7
  DomainControl : Subsystem
  Driver : Subsystem
  Drivetrain : Subsystem
  ElectricalSystem : Subsystem
  Engine : Subsystem
  Environment : Subsystem
  Help : Subsystem
      settings: OpenFcn=eval(get_param(gcb,'MaskHelp'))
      mask Help: asm_modelhelp(0,'tool','ASM_Traffic_lib','ASM_Traffic');
      mask Display: fprintf('Help')
  Terminator{,1..11} (12 alike) : Terminator
  VehicleDynamics : Subsystem
  controller_subsys : Subsystem
  exec_setting : Subsystem
  Out1 : Outport
  wires:
  DomainControl/1(Out) -> BusCreator1/7
  BusCreator1/1 -> ElectricalSystem/1(In), Drivetrain/1(In), Driver/1(In), DomainControl/1(In), AnimationInterface/1(In), Environment/1(In), VehicleDynamics/1(In), Engine/1(In)
  Driver/1(Out) -> BusCreator1/5
  Drivetrain/1(Out) -> BusCreator1/3
  ElectricalSystem/1(Out) -> BusCreator1/1
  Engine/1(Out) -> BusCreator1/2
  Environment/1(Out) -> BusCreator1/6
  VehicleDynamics/1(Out) -> BusCreator1/4
  exec_setting/1(execution) -> controller_subsys/2(execution)  "exec"
  controller_subsys/2(telemetry) -> Bus Selector/1
  controller_subsys/1(command) -> Out1/1
  In Bus Element/1 -> controller_subsys/1(measurements)  "meas_states"
  Bus Selector/1 -> Terminator/1  "<slack_values>"
  Bus Selector/2 -> Terminator1/1  "<solver_status>"
  Bus Selector/3 -> Terminator2/1  "<cost_value>"
  Bus Selector/4 -> Terminator3/1  "<kkt_residuals>"
  Bus Selector/5 -> Terminator4/1  "<cpu_time>"
  Bus Selector/6 -> Terminator5/1  "<cpu_time_qp>"
  Bus Selector/7 -> Terminator6/1  "<cpu_time_lin>"
  Bus Selector/8 -> Terminator7/1  "<sqp_iter>"
  Bus Selector/9 -> Terminator8/1  "<qp_iteration_history>"
  Bus Selector/10 -> Terminator9/1  "<residual_history>"
  Bus Selector/11 -> Terminator10/1  "<history_length>"
  Bus Selector/12 -> Terminator11/1  "<lam_stage0>"
